simulink model "heatdrive_ecc_coupled_se21"  (R2025b)
settings: Solver=ode23t  StartTime=0.0  StopTime=10  FixedStep=0.1  MaxStep=0.4  RelTol=1e-2  AbsTol=1e-3
values from neighbouring files (symbols this model uses):
  cold_load_heat_W = 0.0    (= 0)    [Build_Simulink_Exchange_Params.m]
  cold_load_T_init = get_stage_field(stage_config, 'cold_load_T_in', get_stage_field(stage_config,          'chip_T_in', get_option_field(exchange_options, 'cold_load_T_init', get_option_field(exchange_options, 'chip_T_init', 293.0))))    [Build_Simulink_Exchange_Params.m]    (also in Create_Simulink_Exchange_Runtime.m = get_option_field(options, 'cold_load_T_init',          get_o)
  cold_sink_T_init = get_stage_field(stage_config, 'cold_sink_T_in', get_option_field(exchange_options, 'cold_sink_T_init', 293.0))    [Build_Simulink_Exchange_Params.m]    (also in Create_Simulink_Exchange_Runtime.m = get_option_field(options, 'cold_sink_T_init', ambient_T_init)
  hot_sink_T_init = get_stage_field(stage_config, 'hot_sink_T_in', get_option_field(exchange_options, 'hot_sink_T_init', 293.0))    [Build_Simulink_Exchange_Params.m]    (also in Create_Simulink_Exchange_Runtime.m = get_option_field(options, 'hot_sink_T_init', ambient_T_init))
  mdot_cooldown_source_kgps = mdot_target_kgps    [Build_Simulink_Exchange_Params.m]
  mdot_hold_source_kgps = mdot_target_kgps    [Build_Simulink_Exchange_Params.m]
  pressure_pi_bias_MPa = pressure_pi_dp_guess_MPa    [Build_Simulink_Exchange_Params.m]
  pressure_pi_error_filter_tau_s = max(get_option_field(exchange_options, 'pressure_pi_error_filter_tau_s', 0.002), 1.0e-5)    [Build_Simulink_Exchange_Params.m]
  pressure_pi_error_normalization_gain_kgps_inv = 1.0    (= 1)    [Build_Simulink_Exchange_Params.m]
  pressure_pi_max_MPa = pressure_pi_dp_guess_MPa + pressure_pi_margin_MPa    [Build_Simulink_Exchange_Params.m]
  shex_sink_T_init = get_option_field(exchange_options, 'shex_sink_T_init', hot_sink_T_init)    [Build_Simulink_Exchange_Params.m]
undefined symbols (not defined in the file or in its folder): constitutive_sample_time_s, constitutive_state21_initial, se_constitutive_T21_initial, se_pressure_integrator_max_MPa, se_pressure_pi_ki_MPa_per_kgps_s, se_pressure_pi_kp_MPa_per_kgps, se_pressure_pi_min_MPa, se_solver_T_init_21_internal, se_stage2_pressure_integrator_min_MPa, se_stage4_pressure_integrator_min_MPa, sma_constitutive_T21_initial, sma_mdot_stage1_source_kgps, sma_mdot_stage3_source_kgps, sma_pressure_integrator_max_MPa, sma_pressure_integrator_min_MPa, sma_pressure_pi_ki_MPa_per_kgps_s, sma_pressure_pi_kp_MPa_per_kgps, sma_pressure_pi_min_MPa, sma_solver_T_init_21_internal
libraries: fl_lib x484, nesl_utility x232, SimscapeFluids_lib x20
(part 1 of 8)
settings Model: Creator=Yanchenxi  LastModifiedBy=86182
settings RTWCC: GPUComputeCapability=3.5
settings SimscapeCC: ExplicitSolverDiagnosticOptions=none  SimscapeLogType=all  SimscapeLogSimulationStatistics=on  SimscapeLogToSDI=on

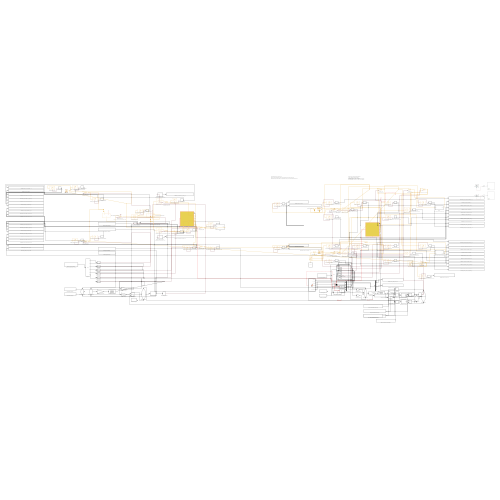
[thumbnail: Simulink's stored preview of the top-level diagram]
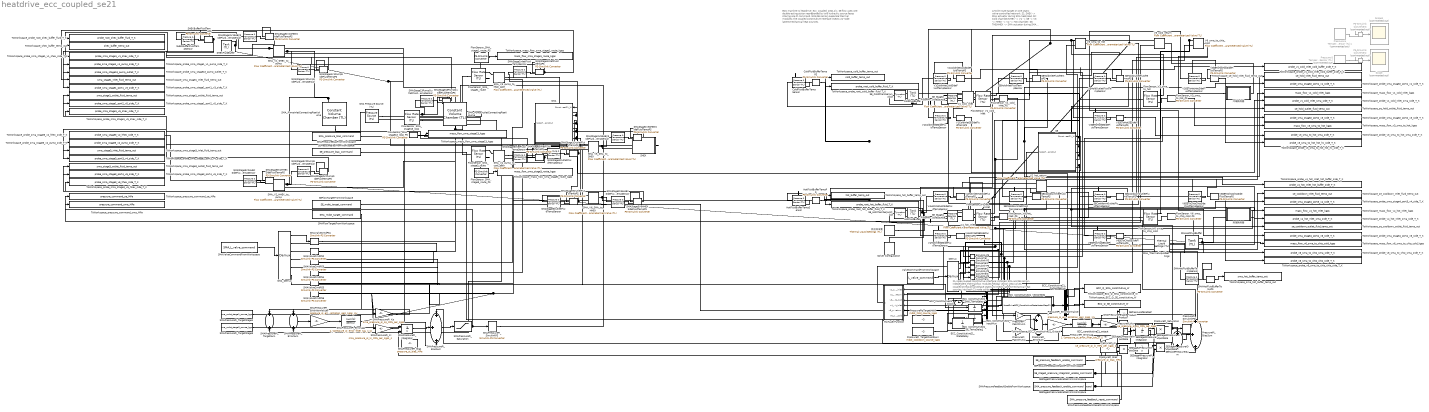
== system heatdrive_ecc_coupled_se21 ==
  note: ECC mainline is heatdrive_ecc_coupled_se21.slx.
      | SE flow uses one double-acting piston represented by two hydraulic source faces sharing one PI command.
      | SMA/SE remain separate thermal modules; the coupled constitutive interface injects 21-node latent/mechanical heat sources.
  note: Article route target on one static valve-controlled network:
      | S1: SHEX -> SMA actuator during SMA heat/load.
      | S2: Cold chamber/CHEX -> V1 -> SE -> V3 -> HHEX -> V2 -> Hot chamber.
      | S3: THE/HHEX -> SMA actuator during SMA cool/unload.
      | S4: Hot chamber/HHEX -> V4 -> SE -> V6 -> CHEX -> V5 -> Cold chamber.
  note: 21-node coupled constitutive interface installed.
      | SMA and SE remain independent thermal/flow modules.
      | Global vector step solves coupled stress/strain/phase state and injects latent/mechanical heat sources into both 21-node solids.
  ColdFluidBuffer : SimscapeFluids_lib/Thermal Liquid/Tanks & Accumulators/Tank (TL)  num_inlet=fluids.thermal_liquid.tanks_accumulators.enum.NumInlet.One  pressure_spec=fluids.thermal_liquid.tanks_accumulators.enum.TankPressureSpec.Specified  tank_pressure=tank_pressure_MPa MPa  volume_spec=fluids.thermal_liquid.tanks_accumulators.enum.TankVolumeSpec.Constant  tank_area=fluid_buffer_tank_area_m2 m^2  level_TLU=[0, 3, 5] m  volume_TLU=[0, 4, 6] m^3  inlet_height_A=0 m  inlet_area_A=0.01 m^2  inlet_heights_AB=[.1, .1] m  inlet_areas_AB=[.01, .01] m^2  inlet_heights_ABC=[.1, .1, .1] m  inlet_areas_ABC=[.01, .01, .01] m^2  inlet_heights_ABCD=0.1 * ones(1, 4) m  inlet_areas_ABCD=0.01 * ones(1, 4) m^2  inlet_heights_ABCDE=0.1 * ones(1, 5) m  inlet_areas_ABCDE=0.01 * ones(1, 5) m^2  inlet_heights_ABCDEF=0.1 * ones(1, 6) m  inlet_areas_ABCDEF=0.01 * ones(1, 6) m^2  level_check=simscape.enum.assert.action.error  capacity_check=simscape.enum.assert.action.none  max_capacity=fluid_buffer_max_capacity_m3 m^3  g=9.81 m/s^2  level_specify=on  level_priority=High  level=fluid_buffer_tank_level_m m  level_nominal_specify=off  level_nominal_value=1  level_nominal_unit=m  volume_specify=off  volume_priority=None  volume=5 m^3  volume_nominal_specify=off  volume_nominal_value=1  volume_nominal_unit=m^3  mass_specify=off  mass_priority=None  mass=5000 kg  mass_nominal_specify=off  mass_nominal_value=1  mass_nominal_unit=kg  T_I_specify=on  T_I_priority=High  T_I=cold_fluid_buffer_T_init K  T_I_nominal_specify=off  T_I_nominal_value=1  T_I_nominal_unit=K
      settings: InternalSimscapePortConfiguration="{\"Bottom\":[{\"id\":\"H\",\"label\":\"H\",\"type\":\"foundation.thermal.thermal\"},{\"id\":\"T_out\",\"label\":\"T\",\"type\":\"output\"}],\"Left\":[{\"id\":\"A\",\"label\":\"A\",\"type\":\"foundation.thermal_liquid.thermal_liquid\"}],\"Right\":[],\"Top\":[{\"id\":\"V_out\",\"label\":\"V\",\"type\":\"output\"},{\"id\":\"L_out\",\"label\":\"L\",\"type\":\"output\"}]}"
  ColdFluidBufferTempPS : nesl_utility/PS-Simulink Converter  PhysicalDomain=network_engine_domain  SubClassName=ps_output  LeftPortType=input  RightPortType=output  PseudoPeriodic=off  Frequencies=[]  VectorFormat=1-D array  Unit=K  AffineConversion=off
      settings: AttributesFormatString=CHEX exchanger retained from mature model
  ColdFluidBufferTempSensor : fl_lib/Thermal Liquid/Sensors/Pressure & Temperature Sensor (TL)  reference=foundation.enum.MeasurementReference.absolute  pressure=false  pressure_spec=foundation.enum.PressureMeasementSpec.Absolute  temperature=true
      settings: InternalSimscapePortConfiguration="{\"Bottom\":[{\"id\":\"T\",\"label\":\"T\",\"type\":\"output\"}],\"Left\":[{\"id\":\"A\",\"label\":\"A\",\"type\":\"foundation.thermal_liquid.thermal_liquid\"}],\"Right\":[],\"Top\":[]}"
  Demux : Demux  Outputs=6
      settings: DisplayOption=none
  ECC_Constitutive21_Clock : Clock
  ECC_Constitutive21_InputMux : Mux
  ECC_Constitutive21_OutputDemux : Demux  Outputs=[21 21 210]
  ECC_Constitutive21_SE_TempDelay : UnitDelay  InitialCondition=se_constitutive_T21_initial  SampleTime=constitutive_sample_time_s  HasFrameUpgradeWarning=on
  ECC_Constitutive21_SMA_TempDelay : UnitDelay  InitialCondition=sma_constitutive_T21_initial  SampleTime=constitutive_sample_time_s  HasFrameUpgradeWarning=on
  ECC_Constitutive21_StateDelay : UnitDelay  InitialCondition=constitutive_state21_initial  SampleTime=constitutive_sample_time_s  HasFrameUpgradeWarning=on
  ECC_Constitutive21_VectorStep : MATLABFcn  MATLABFcn=HeatDriveECC_ConstitutiveStateVectorStep21  OutputDimensions=252  SampleTime=constitutive_sample_time_s
  FlowSensor_SMA_stage13_loop : fl_lib/Thermal Liquid/Sensors/Flow Rate Sensor (TL)  mass_flow_measure=true  volumetric_flow_measure=false  energy_flow_measure=false
      settings: InternalSimscapePortConfiguration="{\"Bottom\":[],\"Left\":[{\"id\":\"A\",\"label\":\"A\",\"type\":\"foundation.thermal_liquid.thermal_liquid\"}],\"Right\":[{\"id\":\"B\",\"label\":\"B\",\"type\":\"foundation.thermal_liquid.thermal_liquid\"},{\"id\":\"M\",\"label\":\"M\",\"type\":\"output\"}],\"Top\":[]}"
  FlowSensor_SMA_stage13_loop_PS : nesl_utility/PS-Simulink Converter  PhysicalDomain=network_engine_domain  SubClassName=ps_output  LeftPortType=input  RightPortType=output  PseudoPeriodic=off  Frequencies=[]  VectorFormat=1-D array  Unit=kg/s  AffineConversion=off
      settings: AttributesFormatString=CHEX exchanger retained from mature model
  FlowSensor_SMA_stage1_route : fl_lib/Thermal Liquid/Sensors/Flow Rate Sensor (TL)  mass_flow_measure=true  volumetric_flow_measure=false  energy_flow_measure=false
      settings: InternalSimscapePortConfiguration="{\"Bottom\":[],\"Left\":[{\"id\":\"A\",\"label\":\"A\",\"type\":\"foundation.thermal_liquid.thermal_liquid\"}],\"Right\":[{\"id\":\"B\",\"label\":\"B\",\"type\":\"foundation.thermal_liquid.thermal_liquid\"},{\"id\":\"M\",\"label\":\"M\",\"type\":\"output\"}],\"Top\":[]}"
  FlowSensor_SMA_stage1_route_PS : nesl_utility/PS-Simulink Converter  PhysicalDomain=network_engine_domain  SubClassName=ps_output  LeftPortType=input  RightPortType=output  PseudoPeriodic=off  Frequencies=[]  VectorFormat=1-D array  Unit=kg/s  AffineConversion=off
      settings: AttributesFormatString=CHEX exchanger retained from mature model
  FlowSensor_SMA_stage3_route : fl_lib/Thermal Liquid/Sensors/Flow Rate Sensor (TL)  mass_flow_measure=true  volumetric_flow_measure=false  energy_flow_measure=false
      settings: InternalSimscapePortConfiguration="{\"Bottom\":[],\"Left\":[{\"id\":\"A\",\"label\":\"A\",\"type\":\"foundation.thermal_liquid.thermal_liquid\"}],\"Right\":[{\"id\":\"B\",\"label\":\"B\",\"type\":\"foundation.thermal_liquid.thermal_liquid\"},{\"id\":\"M\",\"label\":\"M\",\"type\":\"output\"}],\"Top\":[]}"
  FlowSensor_SMA_stage3_route_PS : nesl_utility/PS-Simulink Converter  PhysicalDomain=network_engine_domain  SubClassName=ps_output  LeftPortType=input  RightPortType=output  PseudoPeriodic=off  Frequencies=[]  VectorFormat=1-D array  Unit=kg/s  AffineConversion=off
      settings: AttributesFormatString=CHEX exchanger retained from mature model
  FlowSensor_V1_cold_inlet : fl_lib/Thermal Liquid/Sensors/Flow Rate Sensor (TL)  mass_flow_measure=true  volumetric_flow_measure=false  energy_flow_measure=false
      settings: InternalSimscapePortConfiguration="{\"Bottom\":[],\"Left\":[{\"id\":\"A\",\"label\":\"A\",\"type\":\"foundation.thermal_liquid.thermal_liquid\"}],\"Right\":[{\"id\":\"B\",\"label\":\"B\",\"type\":\"foundation.thermal_liquid.thermal_liquid\"},{\"id\":\"M\",\"label\":\"M\",\"type\":\"output\"}],\"Top\":[]}"
  FlowSensor_V1_cold_inlet_PS : nesl_utility/PS-Simulink Converter  PhysicalDomain=network_engine_domain  SubClassName=ps_output  LeftPortType=input  RightPortType=output  PseudoPeriodic=off  Frequencies=[]  VectorFormat=1-D array  Unit=kg/s  AffineConversion=off
      settings: AttributesFormatString=CHEX exchanger retained from mature model
  FlowSensor_V3_sma_to_hot : fl_lib/Thermal Liquid/Sensors/Flow Rate Sensor (TL)  mass_flow_measure=true  volumetric_flow_measure=false  energy_flow_measure=false
      settings: InternalSimscapePortConfiguration="{\"Bottom\":[],\"Left\":[{\"id\":\"A\",\"label\":\"A\",\"type\":\"foundation.thermal_liquid.thermal_liquid\"}],\"Right\":[{\"id\":\"B\",\"label\":\"B\",\"type\":\"foundation.thermal_liquid.thermal_liquid\"},{\"id\":\"M\",\"label\":\"M\",\"type\":\"output\"}],\"Top\":[]}"
  FlowSensor_V3_sma_to_hot_PS : nesl_utility/PS-Simulink Converter  PhysicalDomain=network_engine_domain  SubClassName=ps_output  LeftPortType=input  RightPortType=output  PseudoPeriodic=off  Frequencies=[]  VectorFormat=1-D array  Unit=kg/s  AffineConversion=off
      settings: AttributesFormatString=HHEX/THE exchanger retained from mature model
  FlowSensor_V4_hot_inlet : fl_lib/Thermal Liquid/Sensors/Flow Rate Sensor (TL)  mass_flow_measure=true  volumetric_flow_measure=false  energy_flow_measure=false
      settings: InternalSimscapePortConfiguration="{\"Bottom\":[],\"Left\":[{\"id\":\"A\",\"label\":\"A\",\"type\":\"foundation.thermal_liquid.thermal_liquid\"}],\"Right\":[{\"id\":\"B\",\"label\":\"B\",\"type\":\"foundation.thermal_liquid.thermal_liquid\"},{\"id\":\"M\",\"label\":\"M\",\"type\":\"output\"}],\"Top\":[]}"
  FlowSensor_V4_hot_inlet_PS : nesl_utility/PS-Simulink Converter  PhysicalDomain=network_engine_domain  SubClassName=ps_output  LeftPortType=input  RightPortType=output  PseudoPeriodic=off  Frequencies=[]  VectorFormat=1-D array  Unit=kg/s  AffineConversion=off
      settings: AttributesFormatString=HHEX/THE exchanger retained from mature model
  FlowSensor_V6_sma_to_chip_cold : fl_lib/Thermal Liquid/Sensors/Flow Rate Sensor (TL)  mass_flow_measure=true  volumetric_flow_measure=false  energy_flow_measure=false
      settings: InternalSimscapePortConfiguration="{\"Bottom\":[],\"Left\":[{\"id\":\"A\",\"label\":\"A\",\"type\":\"foundation.thermal_liquid.thermal_liquid\"}],\"Right\":[{\"id\":\"B\",\"label\":\"B\",\"type\":\"foundation.thermal_liquid.thermal_liquid\"},{\"id\":\"M\",\"label\":\"M\",\"type\":\"output\"}],\"Top\":[]}"
  FlowSensor_V6_sma_to_chip_cold_PS : nesl_utility/PS-Simulink Converter  PhysicalDomain=network_engine_domain  SubClassName=ps_output  LeftPortType=input  RightPortType=output  PseudoPeriodic=off  Frequencies=[]  VectorFormat=1-D array  Unit=kg/s  AffineConversion=off
      settings: AttributesFormatString=CHEX exchanger retained from mature model
  HotFluidBuffer : SimscapeFluids_lib/Thermal Liquid/Tanks & Accumulators/Tank (TL)  num_inlet=fluids.thermal_liquid.tanks_accumulators.enum.NumInlet.One  pressure_spec=fluids.thermal_liquid.tanks_accumulators.enum.TankPressureSpec.Specified  tank_pressure=tank_pressure_MPa MPa  volume_spec=fluids.thermal_liquid.tanks_accumulators.enum.TankVolumeSpec.Constant  tank_area=fluid_buffer_tank_area_m2 m^2  level_TLU=[0, 3, 5] m  volume_TLU=[0, 4, 6] m^3  inlet_height_A=0 m  inlet_area_A=0.01 m^2  inlet_heights_AB=[.1, .1] m  inlet_areas_AB=[.01, .01] m^2  inlet_heights_ABC=[.1, .1, .1] m  inlet_areas_ABC=[.01, .01, .01] m^2  inlet_heights_ABCD=0.1 * ones(1, 4) m  inlet_areas_ABCD=0.01 * ones(1, 4) m^2  inlet_heights_ABCDE=0.1 * ones(1, 5) m  inlet_areas_ABCDE=0.01 * ones(1, 5) m^2  inlet_heights_ABCDEF=0.1 * ones(1, 6) m  inlet_areas_ABCDEF=0.01 * ones(1, 6) m^2  level_check=simscape.enum.assert.action.error  capacity_check=simscape.enum.assert.action.none  max_capacity=fluid_buffer_max_capacity_m3 m^3  g=9.81 m/s^2  level_specify=on  level_priority=High  level=fluid_buffer_tank_level_m m  level_nominal_specify=off  level_nominal_value=1  level_nominal_unit=m  volume_specify=off  volume_priority=None  volume=5 m^3  volume_nominal_specify=off  volume_nominal_value=1  volume_nominal_unit=m^3  mass_specify=off  mass_priority=None  mass=5000 kg  mass_nominal_specify=off  mass_nominal_value=1  mass_nominal_unit=kg  T_I_specify=on  T_I_priority=High  T_I=hot_fluid_buffer_T_init K  T_I_nominal_specify=off  T_I_nominal_value=1  T_I_nominal_unit=K
      settings: InternalSimscapePortConfiguration="{\"Bottom\":[{\"id\":\"H\",\"label\":\"H\",\"type\":\"foundation.thermal.thermal\"},{\"id\":\"T_out\",\"label\":\"T\",\"type\":\"output\"}],\"Left\":[{\"id\":\"A\",\"label\":\"A\",\"type\":\"foundation.thermal_liquid.thermal_liquid\"}],\"Right\":[],\"Top\":[{\"id\":\"V_out\",\"label\":\"V\",\"type\":\"output\"},{\"id\":\"L_out\",\"label\":\"L\",\"type\":\"output\"}]}"
  HotFluidBufferTempPS : nesl_utility/PS-Simulink Converter  PhysicalDomain=network_engine_domain  SubClassName=ps_output  LeftPortType=input  RightPortType=output  PseudoPeriodic=off  Frequencies=[]  VectorFormat=1-D array  Unit=K  AffineConversion=off
      settings: AttributesFormatString=HHEX/THE exchanger retained from mature model
  HotFluidBufferTempSensor : fl_lib/Thermal Liquid/Sensors/Pressure & Temperature Sensor (TL)  reference=foundation.enum.MeasurementReference.absolute  pressure=false  pressure_spec=foundation.enum.PressureMeasementSpec.Absolute  temperature=true
      settings: InternalSimscapePortConfiguration="{\"Bottom\":[{\"id\":\"T\",\"label\":\"T\",\"type\":\"output\"}],\"Left\":[{\"id\":\"A\",\"label\":\"A\",\"type\":\"foundation.thermal_liquid.thermal_liquid\"}],\"Right\":[],\"Top\":[]}"
  MATLAB Function : MATLAB Function  TreatAsAtomicUnit=on
  PS-Simulink Converter2 : nesl_utility/PS-Simulink Converter  Commented=on  PhysicalDomain=network_engine_domain  SubClassName=ps_output  LeftPortType=input  RightPortType=output  PseudoPeriodic=off  Frequencies=[]  VectorFormat=1-D array  Unit=1  AffineConversion=off
  PS-Simulink Converter3 : nesl_utility/PS-Simulink Converter  Commented=on  PhysicalDomain=network_engine_domain  SubClassName=ps_output  LeftPortType=input  RightPortType=output  PseudoPeriodic=off  Frequencies=[]  VectorFormat=1-D array  Unit=1  AffineConversion=off
  Pressure & Temperature Sensor (TL) : fl_lib/Thermal Liquid/Sensors/Pressure & Temperature Sensor (TL)  Commented=on  reference=foundation.enum.MeasurementReference.absolute  pressure=false  pressure_spec=foundation.enum.PressureMeasementSpec.Absolute  temperature=true
      settings: InternalSimscapePortConfiguration="{\"Bottom\":[{\"id\":\"T\",\"label\":\"T\",\"type\":\"output\"}],\"Left\":[{\"id\":\"A\",\"label\":\"A\",\"type\":\"foundation.thermal_liquid.thermal_liquid\"}],\"Right\":[],\"Top\":[]}"
  Pressure & Temperature Sensor (TL)1 : fl_lib/Thermal Liquid/Sensors/Pressure & Temperature Sensor (TL)  Commented=on  reference=foundation.enum.MeasurementReference.absolute  pressure=false  pressure_spec=foundation.enum.PressureMeasementSpec.Absolute  temperature=true
      settings: InternalSimscapePortConfiguration="{\"Bottom\":[{\"id\":\"T\",\"label\":\"T\",\"type\":\"output\"}],\"Left\":[{\"id\":\"A\",\"label\":\"A\",\"type\":\"foundation.thermal_liquid.thermal_liquid\"}],\"Right\":[],\"Top\":[]}"
  PressurePI_Bias : Constant  Value=pressure_pi_bias_MPa
  PressurePI_BiasSum : Sum  Inputs=+++
  PressurePI_ErrorLag : TransferFcn  Numerator=1  Denominator=[pressure_pi_error_filter_tau_s 1]
  PressurePI_ErrorNormalizer : Gain  Gain=pressure_pi_error_normalization_gain_kgps_inv
  PressurePI_ErrorSum : Sum  Inputs=++--
  PressurePI_Ki : Gain  Gain=se_pressure_pi_ki_MPa_per_kgps_s
  PressurePI_Kp : Gain  Gain=se_pressure_pi_kp_MPa_per_kgps
  PressurePI_PassthruV1 : Gain
  PressurePI_PassthruV4 : Gain
  PressurePI_Saturation : Saturate  UpperLimit=pressure_pi_max_MPa  LowerLimit=se_pressure_pi_min_MPa
  PressurePI_SimulinkPS : nesl_utility/Simulink-PS Converter  PhysicalDomain=network_engine_domain  SubClassName=ps_input  LeftPortType=input  RightPortType=output  PseudoPeriodic=off  Frequencies=[]  NoiseDistribution=none  NoiseParameters=[]  Unit=MPa  AffineConversion=off  FilteringAndDerivatives=provide  SimscapeFilterOrder=1  InputFilterTimeConstant=0.001  UdotUserProvided=0
  PressurePI_TargetCooldown : Constant  Value=mdot_cooldown_source_kgps
  PressurePI_TargetHold : Constant  Value=mdot_hold_source_kgps
  SE : Subsystem
      settings: AttributesFormatString=Active dual-path SE21 exchanger shell; ECC solid law is handled separately
  SECooldownInletFluidTempPS : nesl_utility/PS-Simulink Converter  PhysicalDomain=network_engine_domain  SubClassName=ps_output  LeftPortType=input  RightPortType=output  PseudoPeriodic=off  Frequencies=[]  VectorFormat=1-D array  Unit=K  AffineConversion=off
  SECooldownInletFluidTempSensor : fl_lib/Thermal Liquid/Sensors/Pressure & Temperature Sensor (TL)  reference=foundation.enum.MeasurementReference.absolute  pressure=false  pressure_spec=foundation.enum.PressureMeasementSpec.Absolute  temperature=true
      settings: InternalSimscapePortConfiguration="{\"Bottom\":[{\"id\":\"T\",\"label\":\"T\",\"type\":\"output\"}],\"Left\":[{\"id\":\"A\",\"label\":\"A\",\"type\":\"foundation.thermal_liquid.thermal_liquid\"}],\"Right\":[],\"Top\":[]}"
  SECooldownOutletFluidTempPS : nesl_utility/PS-Simulink Converter  PhysicalDomain=network_engine_domain  SubClassName=ps_output  LeftPortType=input  RightPortType=output  PseudoPeriodic=off  Frequencies=[]  VectorFormat=1-D array  Unit=K  AffineConversion=off
  SECooldownOutletFluidTempSensor : fl_lib/Thermal Liquid/Sensors/Pressure & Temperature Sensor (TL)  reference=foundation.enum.MeasurementReference.absolute  pressure=false  pressure_spec=foundation.enum.PressureMeasementSpec.Absolute  temperature=true
      settings: InternalSimscapePortConfiguration="{\"Bottom\":[{\"id\":\"T\",\"label\":\"T\",\"type\":\"output\"}],\"Left\":[{\"id\":\"A\",\"label\":\"A\",\"type\":\"foundation.thermal_liquid.thermal_liquid\"}],\"Right\":[],\"Top\":[]}"
  SEFlowTargetFromWorkspace : FromWorkspace  VariableName=SE_mdot_target_command  OutputAfterFinalValue=Holding final value
  SEHoldInletFluidTempPS : nesl_utility/PS-Simulink Converter  PhysicalDomain=network_engine_domain  SubClassName=ps_output  LeftPortType=input  RightPortType=output  PseudoPeriodic=off  Frequencies=[]  VectorFormat=1-D array  Unit=K  AffineConversion=off
  SEHoldInletFluidTempSensor : fl_lib/Thermal Liquid/Sensors/Pressure & Temperature Sensor (TL)  reference=foundation.enum.MeasurementReference.absolute  pressure=false  pressure_spec=foundation.enum.PressureMeasementSpec.Absolute  temperature=true
      settings: InternalSimscapePortConfiguration="{\"Bottom\":[{\"id\":\"T\",\"label\":\"T\",\"type\":\"output\"}],\"Left\":[{\"id\":\"A\",\"label\":\"A\",\"type\":\"foundation.thermal_liquid.thermal_liquid\"}],\"Right\":[],\"Top\":[]}"
  SEHoldOutletFluidTempPS : nesl_utility/PS-Simulink Converter  PhysicalDomain=network_engine_domain  SubClassName=ps_output  LeftPortType=input  RightPortType=output  PseudoPeriodic=off  Frequencies=[]  VectorFormat=1-D array  Unit=K  AffineConversion=off
  SEHoldOutletFluidTempSensor : fl_lib/Thermal Liquid/Sensors/Pressure & Temperature Sensor (TL)  reference=foundation.enum.MeasurementReference.absolute  pressure=false  pressure_spec=foundation.enum.PressureMeasementSpec.Absolute  temperature=true
      settings: InternalSimscapePortConfiguration="{\"Bottom\":[{\"id\":\"T\",\"label\":\"T\",\"type\":\"output\"}],\"Left\":[{\"id\":\"A\",\"label\":\"A\",\"type\":\"foundation.thermal_liquid.thermal_liquid\"}],\"Right\":[],\"Top\":[]}"
  SEPressureBiasFromWorkspace : FromWorkspace  VariableName=SE_pressure_bias_command  OutputAfterFinalValue=Holding final value
  SEPressureFeedbackEnableFromWorkspace : FromWorkspace  VariableName=SE_pressure_feedback_enable_command  Interpolate=off  OutputAfterFinalValue=Holding final value
  SEPressurePEnableProduct : Product  Inputs=**
  SERoutePressureISum : Sum
  SEStage2PressureIEnableFromWorkspace : FromWorkspace  VariableName=SE_stage2_pressure_integrator_enable_command  Interpolate=off  OutputAfterFinalValue=Holding final value
  SEStage2PressureIInputGate : Product  Inputs=**
  SEStage2PressureIOutputGate : Product  Inputs=**
  SEStage2PressurePI_Integrator : Integrator  LimitOutput=on  UpperSaturationLimit=se_pressure_integrator_max_MPa  LowerSaturationLimit=se_stage2_pressure_integrator_min_MPa
  SEStage4PressureIEnableFromWorkspace : FromWorkspace  VariableName=SE_stage4_pressure_integrator_enable_command  Interpolate=off  OutputAfterFinalValue=Holding final value
  SEStage4PressureIInputGate : Product  Inputs=**
  SEStage4PressureIOutputGate : Product  Inputs=**
  SEStage4PressurePI_Integrator : Integrator  LimitOutput=on  UpperSaturationLimit=se_pressure_integrator_max_MPa  LowerSaturationLimit=se_stage4_pressure_integrator_min_MPa
  SE_ColdChamberJunction : SimscapeFluids_lib/Thermal Liquid/Pipes & Fittings/T-Junction (TL)  area_main=pipe_fa m^2  area_branch=pipe_fa m^2  junction_spec=fluids.thermal_liquid.pipes_fittings.enum.TLossCoefficientModel.Crane  k_main_converge=1.12  k_main_diverge=1.12  k_branch_converge=1.12  k_branch_diverge=1.12  loss_coeff_A=1  loss_coeff_B=1  loss_coeff_C=1  radius=0.001 m  Re_c=150  Re_0=10  tau=0.0001 s  saturation_ratio=0.2  smoothing_factor=0.01  inertia=false
      settings: InternalSimscapePortConfiguration="{\"Bottom\":[{\"id\":\"C\",\"label\":\"C\",\"type\":\"foundation.thermal_liquid.thermal_liquid\"}],\"Left\":[{\"id\":\"A\",\"label\":\"A\",\"type\":\"foundation.thermal_liquid.thermal_liquid\"}],\"Right\":[{\"id\":\"B\",\"label\":\"B\",\"type\":\"foundation.thermal_liquid.thermal_liquid\"}],\"Top\":[]}"
  SE_HotChamberJunction : SimscapeFluids_lib/Thermal Liquid/Pipes & Fittings/T-Junction (TL)  area_main=0.01 m^2  area_branch=0.01 m^2  junction_spec=fluids.thermal_liquid.pipes_fittings.enum.TLossCoefficientModel.Crane  k_main_converge=1.12  k_main_diverge=1.12  k_branch_converge=1.12  k_branch_diverge=1.12  loss_coeff_A=1  loss_coeff_B=1  loss_coeff_C=1  radius=0.001 m  Re_c=150  Re_0=10  tau=0.0001 s  saturation_ratio=0.2  smoothing_factor=0.01  inertia=false
      settings: InternalSimscapePortConfiguration="{\"Bottom\":[{\"id\":\"C\",\"label\":\"C\",\"type\":\"foundation.thermal_liquid.thermal_liquid\"}],\"Left\":[{\"id\":\"A\",\"label\":\"A\",\"type\":\"foundation.thermal_liquid.thermal_liquid\"}],\"Right\":[{\"id\":\"B\",\"label\":\"B\",\"type\":\"foundation.thermal_liquid.thermal_liquid\"}],\"Top\":[]}"
  SE_Stage2_PistonPressureSource : fl_lib/Thermal Liquid/Sources/Pressure Source (TL)  source_type=foundation.enum.constant_controlled.controlled  pressure_differential=pressure_differential_MPa MPa  power_spec=foundation.enum.power_spec.none  area=pipe_fa m^2
      settings: AttributesFormatString=Stage 2 hydraulic face of the single SE double-acting piston  InternalSimscapePortConfiguration="{\"Bottom\":[],\"Left\":[{\"id\":\"A\",\"label\":\"A\",\"type\":\"foundation.thermal_liquid.thermal_liquid\"},{\"id\":\"P\",\"label\":\"P\",\"type\":\"input\"}],\"Right\":[{\"id\":\"B\",\"label\":\"B\",\"type\":\"foundation.thermal_liquid.thermal_liquid\"}],\"Top\":[]}"
  SE_Stage4_PistonPressureSource : fl_lib/Thermal Liquid/Sources/Pressure Source (TL)  source_type=foundation.enum.constant_controlled.controlled  pressure_differential=pressure_differential_MPa MPa  power_spec=foundation.enum.power_spec.none  area=pipe_fa m^2
      settings: AttributesFormatString=Stage 4 hydraulic face of the single SE double-acting piston  InternalSimscapePortConfiguration="{\"Bottom\":[],\"Left\":[{\"id\":\"A\",\"label\":\"A\",\"type\":\"foundation.thermal_liquid.thermal_liquid\"},{\"id\":\"P\",\"label\":\"P\",\"type\":\"input\"}],\"Right\":[{\"id\":\"B\",\"label\":\"B\",\"type\":\"foundation.thermal_liquid.thermal_liquid\"}],\"Top\":[]}"
  SHEX : Subsystem
  SHEXBufferFluidTempPS : nesl_utility/PS-Simulink Converter  PhysicalDomain=network_engine_domain  SubClassName=ps_output  LeftPortType=input  RightPortType=output  PseudoPeriodic=off  Frequencies=[]  VectorFormat=1-D array  Unit=K  AffineConversion=off
  SHEXBufferFluidTempSensor : fl_lib/Thermal Liquid/Sensors/Pressure & Temperature Sensor (TL)  reference=foundation.enum.MeasurementReference.absolute  pressure=false  pressure_spec=foundation.enum.PressureMeasementSpec.Absolute  temperature=true
      settings: InternalSimscapePortConfiguration="{\"Bottom\":[{\"id\":\"T\",\"label\":\"T\",\"type\":\"output\"}],\"Left\":[{\"id\":\"A\",\"label\":\"A\",\"type\":\"foundation.thermal_liquid.thermal_liquid\"}],\"Right\":[],\"Top\":[]}"
  SHEXFluidBuffer : SimscapeFluids_lib/Thermal Liquid/Tanks & Accumulators/Tank (TL)  num_inlet=fluids.thermal_liquid.tanks_accumulators.enum.NumInlet.One  pressure_spec=fluids.thermal_liquid.tanks_accumulators.enum.TankPressureSpec.Specified  tank_pressure=tank_pressure_MPa MPa  volume_spec=fluids.thermal_liquid.tanks_accumulators.enum.TankVolumeSpec.Constant  tank_area=fluid_buffer_tank_area_m2 m^2  level_TLU=[0, 3, 5] m  volume_TLU=[0, 4, 6] m^3  inlet_height_A=0 m  inlet_area_A=0.01 m^2  inlet_heights_AB=[.1, .1] m  inlet_areas_AB=[.01, .01] m^2  inlet_heights_ABC=[.1, .1, .1] m  inlet_areas_ABC=[.01, .01, .01] m^2  inlet_heights_ABCD=0.1 * ones(1, 4) m  inlet_areas_ABCD=0.01 * ones(1, 4) m^2  inlet_heights_ABCDE=0.1 * ones(1, 5) m  inlet_areas_ABCDE=0.01 * ones(1, 5) m^2  inlet_heights_ABCDEF=0.1 * ones(1, 6) m  inlet_areas_ABCDEF=0.01 * ones(1, 6) m^2  level_check=simscape.enum.assert.action.error  capacity_check=simscape.enum.assert.action.none  max_capacity=fluid_buffer_max_capacity_m3 m^3  g=9.81 m/s^2  level_specify=on  level_priority=High  level=fluid_buffer_tank_level_m m  level_nominal_specify=off  level_nominal_value=1  level_nominal_unit=m  volume_specify=off  volume_priority=None  volume=5 m^3  volume_nominal_specify=off  volume_nominal_value=1  volume_nominal_unit=m^3  mass_specify=off  mass_priority=None  mass=5000 kg  mass_nominal_specify=off  mass_nominal_value=1  mass_nominal_unit=kg  T_I_specify=on  T_I_priority=High  T_I=shex_fluid_buffer_T_init K  T_I_nominal_specify=off  T_I_nominal_value=1  T_I_nominal_unit=K
      settings: InternalSimscapePortConfiguration="{\"Bottom\":[{\"id\":\"H\",\"label\":\"H\",\"type\":\"foundation.thermal.thermal\"},{\"id\":\"T_out\",\"label\":\"T\",\"type\":\"output\"}],\"Left\":[{\"id\":\"A\",\"label\":\"A\",\"type\":\"foundation.thermal_liquid.thermal_liquid\"}],\"Right\":[],\"Top\":[{\"id\":\"V_out\",\"label\":\"V\",\"type\":\"output\"},{\"id\":\"L_out\",\"label\":\"L\",\"type\":\"output\"}]}"
  SMA : Subsystem
  SMA Pressure Source (TL) : fl_lib/Thermal Liquid/Sources/Pressure Source (TL)  source_type=foundation.enum.constant_controlled.controlled  pressure_differential=pressure_differential_MPa MPa  power_spec=foundation.enum.power_spec.none  area=sma_pipe_fa m^2
      settings: AttributesFormatString=ECC pump / pressure source retained from mature model  InternalSimscapePortConfiguration="{\"Bottom\":[],\"Left\":[{\"id\":\"A\",\"label\":\"A\",\"type\":\"foundation.thermal_liquid.thermal_liquid\"},{\"id\":\"P\",\"label\":\"P\",\"type\":\"input\"}],\"Right\":[{\"id\":\"B\",\"label\":\"B\",\"type\":\"foundation.thermal_liquid.thermal_liquid\"}],\"Top\":[]}"
  SMAFlowTargetFromWorkspace : FromWorkspace  VariableName=SMA_mdot_target_command  OutputAfterFinalValue=Holding final value
  SMAHotFluidBuffer : SimscapeFluids_lib/Thermal Liquid/Tanks & Accumulators/Tank (TL)  num_inlet=fluids.thermal_liquid.tanks_accumulators.enum.NumInlet.One  pressure_spec=fluids.thermal_liquid.tanks_accumulators.enum.TankPressureSpec.Specified  tank_pressure=tank_pressure_MPa MPa  volume_spec=fluids.thermal_liquid.tanks_accumulators.enum.TankVolumeSpec.Constant  tank_area=fluid_buffer_tank_area_m2 m^2  level_TLU=[0, 3, 5] m  volume_TLU=[0, 4, 6] m^3  inlet_height_A=0 m  inlet_area_A=0.01 m^2  inlet_heights_AB=[.1, .1] m  inlet_areas_AB=[.01, .01] m^2  inlet_heights_ABC=[.1, .1, .1] m  inlet_areas_ABC=[.01, .01, .01] m^2  inlet_heights_ABCD=0.1 * ones(1, 4) m  inlet_areas_ABCD=0.01 * ones(1, 4) m^2  inlet_heights_ABCDE=0.1 * ones(1, 5) m  inlet_areas_ABCDE=0.01 * ones(1, 5) m^2  inlet_heights_ABCDEF=0.1 * ones(1, 6) m  inlet_areas_ABCDEF=0.01 * ones(1, 6) m^2  level_check=simscape.enum.assert.action.error  capacity_check=simscape.enum.assert.action.none  max_capacity=fluid_buffer_max_capacity_m3 m^3  g=9.81 m/s^2  level_specify=on  level_priority=High  level=fluid_buffer_tank_level_m m  level_nominal_specify=off  level_nominal_value=1  level_nominal_unit=m  volume_specify=off  volume_priority=None  volume=5 m^3  volume_nominal_specify=off  volume_nominal_value=1  volume_nominal_unit=m^3  mass_specify=off  mass_priority=None  mass=5000 kg  mass_nominal_specify=off  mass_nominal_value=1  mass_nominal_unit=kg  T_I_specify=on  T_I_priority=High  T_I=hot_fluid_buffer_T_init K  T_I_nominal_specify=off  T_I_nominal_value=1  T_I_nominal_unit=K
      settings: InternalSimscapePortConfiguration="{\"Bottom\":[{\"id\":\"H\",\"label\":\"H\",\"type\":\"foundation.thermal.thermal\"},{\"id\":\"T_out\",\"label\":\"T\",\"type\":\"output\"}],\"Left\":[{\"id\":\"A\",\"label\":\"A\",\"type\":\"foundation.thermal_liquid.thermal_liquid\"}],\"Right\":[],\"Top\":[{\"id\":\"V_out\",\"label\":\"V\",\"type\":\"output\"},{\"id\":\"L_out\",\"label\":\"L\",\"type\":\"output\"}]}"
  SMAHotFluidBufferTempPS : nesl_utility/PS-Simulink Converter  PhysicalDomain=network_engine_domain  SubClassName=ps_output  LeftPortType=input  RightPortType=output  PseudoPeriodic=off  Frequencies=[]  VectorFormat=1-D array  Unit=K  AffineConversion=off
      settings: AttributesFormatString=HHEX/THE exchanger retained from mature model
  SMAHotFluidBufferTempSensor : fl_lib/Thermal Liquid/Sensors/Pressure & Temperature Sensor (TL)  reference=foundation.enum.MeasurementReference.absolute  pressure=false  pressure_spec=foundation.enum.PressureMeasementSpec.Absolute  temperature=true
      settings: InternalSimscapePortConfiguration="{\"Bottom\":[{\"id\":\"T\",\"label\":\"T\",\"type\":\"output\"}],\"Left\":[{\"id\":\"A\",\"label\":\"A\",\"type\":\"foundation.thermal_liquid.thermal_liquid\"}],\"Right\":[],\"Top\":[]}"
  SMAPressureBiasFromWorkspace : FromWorkspace  VariableName=SMA_pressure_bias_command  OutputAfterFinalValue=Holding final value
  SMAPressureFeedbackEnableFromWorkspace : FromWorkspace  VariableName=SMA_pressure_feedback_enable_command  Interpolate=off  OutputAfterFinalValue=Holding final value
  SMAPressureFeedbackResetFromWorkspace : FromWorkspace  VariableName=SMA_pressure_feedback_reset_command  Interpolate=off  OutputAfterFinalValue=Holding final value
  SMAPressurePEnableProduct : Product  Inputs=**
  SMAPressurePI_Bias : Constant  Value=pressure_pi_bias_MPa
  SMAPressurePI_BiasSum : Sum  Inputs=+++
  SMAPressurePI_ErrorLag : TransferFcn  Numerator=1  Denominator=[pressure_pi_error_filter_tau_s 1]
  SMAPressurePI_ErrorNormalizer : Gain  Gain=pressure_pi_error_normalization_gain_kgps_inv
  SMAPressurePI_ErrorSum : Sum
  SMAPressurePI_Integrator : Integrator  ExternalReset=level  LimitOutput=on  UpperSaturationLimit=sma_pressure_integrator_max_MPa  LowerSaturationLimit=sma_pressure_integrator_min_MPa
  SMAPressurePI_Ki : Gain  Gain=sma_pressure_pi_ki_MPa_per_kgps_s
  SMAPressurePI_Kp : Gain  Gain=sma_pressure_pi_kp_MPa_per_kgps
  SMAPressurePI_Saturation : Saturate  UpperLimit=pressure_pi_max_MPa  LowerLimit=sma_pressure_pi_min_MPa
  SMAPressurePI_SimulinkPS : nesl_utility/Simulink-PS Converter  PhysicalDomain=network_engine_domain  SubClassName=ps_input  LeftPortType=input  RightPortType=output  PseudoPeriodic=off  Frequencies=[]  NoiseDistribution=none  NoiseParameters=[]  Unit=MPa  AffineConversion=off  FilteringAndDerivatives=provide  SimscapeFilterOrder=1  InputFilterTimeConstant=0.001  UdotUserProvided=0
  SMAPressurePI_TargetStage1 : Constant  Value=sma_mdot_stage1_source_kgps
  SMAPressurePI_TargetStage3 : Constant  Value=sma_mdot_stage3_source_kgps
  SMAPressurePI_TargetSum : Sum
  SMAStage13PumpOutletFluidTempPS : nesl_utility/PS-Simulink Converter  PhysicalDomain=network_engine_domain  SubClassName=ps_output  LeftPortType=input  RightPortType=output  PseudoPeriodic=off  Frequencies=[]  VectorFormat=1-D array  Unit=K  AffineConversion=off
  SMAStage13PumpOutletFluidTempSensor : fl_lib/Thermal Liquid/Sensors/Pressure & Temperature Sensor (TL)  reference=foundation.enum.MeasurementReference.absolute  pressure=false  pressure_spec=foundation.enum.PressureMeasementSpec.Absolute  temperature=true
      settings: InternalSimscapePortConfiguration="{\"Bottom\":[{\"id\":\"T\",\"label\":\"T\",\"type\":\"output\"}],\"Left\":[{\"id\":\"A\",\"label\":\"A\",\"type\":\"foundation.thermal_liquid.thermal_liquid\"}],\"Right\":[],\"Top\":[]}"
  SMAStage1InletFluidTempPS : nesl_utility/PS-Simulink Converter  PhysicalDomain=network_engine_domain  SubClassName=ps_output  LeftPortType=input  RightPortType=output  PseudoPeriodic=off  Frequencies=[]  VectorFormat=1-D array  Unit=K  AffineConversion=off
  SMAStage1InletFluidTempSensor : fl_lib/Thermal Liquid/Sensors/Pressure & Temperature Sensor (TL)  reference=foundation.enum.MeasurementReference.absolute  pressure=false  pressure_spec=foundation.enum.PressureMeasementSpec.Absolute  temperature=true
      settings: InternalSimscapePortConfiguration="{\"Bottom\":[{\"id\":\"T\",\"label\":\"T\",\"type\":\"output\"}],\"Left\":[{\"id\":\"A\",\"label\":\"A\",\"type\":\"foundation.thermal_liquid.thermal_liquid\"}],\"Right\":[],\"Top\":[]}"
  SMAStage1OutletFluidTempPS : nesl_utility/PS-Simulink Converter  PhysicalDomain=network_engine_domain  SubClassName=ps_output  LeftPortType=input  RightPortType=output  PseudoPeriodic=off  Frequencies=[]  VectorFormat=1-D array  Unit=K  AffineConversion=off
  SMAStage1OutletFluidTempSensor : fl_lib/Thermal Liquid/Sensors/Pressure & Temperature Sensor (TL)  reference=foundation.enum.MeasurementReference.absolute  pressure=false  pressure_spec=foundation.enum.PressureMeasementSpec.Absolute  temperature=true
      settings: InternalSimscapePortConfiguration="{\"Bottom\":[{\"id\":\"T\",\"label\":\"T\",\"type\":\"output\"}],\"Left\":[{\"id\":\"A\",\"label\":\"A\",\"type\":\"foundation.thermal_liquid.thermal_liquid\"}],\"Right\":[],\"Top\":[]}"
  SMAStage1V1PumpSideFluidTempPS : nesl_utility/PS-Simulink Converter  PhysicalDomain=network_engine_domain  SubClassName=ps_output  LeftPortType=input  RightPortType=output  PseudoPeriodic=off  Frequencies=[]  VectorFormat=1-D array  Unit=K  AffineConversion=off
  SMAStage1V1PumpSideFluidTempSensor : fl_lib/Thermal Liquid/Sensors/Pressure & Temperature Sensor (TL)  reference=foundation.enum.MeasurementReference.absolute  pressure=false  pressure_spec=foundation.enum.PressureMeasementSpec.Absolute  temperature=true
      settings: InternalSimscapePortConfiguration="{\"Bottom\":[{\"id\":\"T\",\"label\":\"T\",\"type\":\"output\"}],\"Left\":[{\"id\":\"A\",\"label\":\"A\",\"type\":\"foundation.thermal_liquid.thermal_liquid\"}],\"Right\":[],\"Top\":[]}"
  SMAStage1V1SHEXSideFluidTempPS : nesl_utility/PS-Simulink Converter  PhysicalDomain=network_engine_domain  SubClassName=ps_output  LeftPortType=input  RightPortType=output  PseudoPeriodic=off  Frequencies=[]  VectorFormat=1-D array  Unit=K  AffineConversion=off
  SMAStage1V1SHEXSideFluidTempSensor : fl_lib/Thermal Liquid/Sensors/Pressure & Temperature Sensor (TL)  reference=foundation.enum.MeasurementReference.absolute  pressure=false  pressure_spec=foundation.enum.PressureMeasementSpec.Absolute  temperature=true
      settings: InternalSimscapePortConfiguration="{\"Bottom\":[{\"id\":\"T\",\"label\":\"T\",\"type\":\"output\"}],\"Left\":[{\"id\":\"A\",\"label\":\"A\",\"type\":\"foundation.thermal_liquid.thermal_liquid\"}],\"Right\":[],\"Top\":[]}"
  SMAStage1V5SHEXSideFluidTempPS : nesl_utility/PS-Simulink Converter  PhysicalDomain=network_engine_domain  SubClassName=ps_output  LeftPortType=input  RightPortType=output  PseudoPeriodic=off  Frequencies=[]  VectorFormat=1-D array  Unit=K  AffineConversion=off
  SMAStage1V5SHEXSideFluidTempSensor : fl_lib/Thermal Liquid/Sensors/Pressure & Temperature Sensor (TL)  reference=foundation.enum.MeasurementReference.absolute  pressure=false  pressure_spec=foundation.enum.PressureMeasementSpec.Absolute  temperature=true
      settings: InternalSimscapePortConfiguration="{\"Bottom\":[{\"id\":\"T\",\"label\":\"T\",\"type\":\"output\"}],\"Left\":[{\"id\":\"A\",\"label\":\"A\",\"type\":\"foundation.thermal_liquid.thermal_liquid\"}],\"Right\":[],\"Top\":[]}"
  SMAStage3InletFluidTempPS : nesl_utility/PS-Simulink Converter  PhysicalDomain=network_engine_domain  SubClassName=ps_output  LeftPortType=input  RightPortType=output  PseudoPeriodic=off  Frequencies=[]  VectorFormat=1-D array  Unit=K  AffineConversion=off
  SMAStage3InletFluidTempSensor : fl_lib/Thermal Liquid/Sensors/Pressure & Temperature Sensor (TL)  reference=foundation.enum.MeasurementReference.absolute  pressure=false  pressure_spec=foundation.enum.PressureMeasementSpec.Absolute  temperature=true
      settings: InternalSimscapePortConfiguration="{\"Bottom\":[{\"id\":\"T\",\"label\":\"T\",\"type\":\"output\"}],\"Left\":[{\"id\":\"A\",\"label\":\"A\",\"type\":\"foundation.thermal_liquid.thermal_liquid\"}],\"Right\":[],\"Top\":[]}"
  SMAStage3OutletFluidTempPS : nesl_utility/PS-Simulink Converter  PhysicalDomain=network_engine_domain  SubClassName=ps_output  LeftPortType=input  RightPortType=output  PseudoPeriodic=off  Frequencies=[]  VectorFormat=1-D array  Unit=K  AffineConversion=off
  SMAStage3OutletFluidTempSensor : fl_lib/Thermal Liquid/Sensors/Pressure & Temperature Sensor (TL)  reference=foundation.enum.MeasurementReference.absolute  pressure=false  pressure_spec=foundation.enum.PressureMeasementSpec.Absolute  temperature=true
      settings: InternalSimscapePortConfiguration="{\"Bottom\":[{\"id\":\"T\",\"label\":\"T\",\"type\":\"output\"}],\"Left\":[{\"id\":\"A\",\"label\":\"A\",\"type\":\"foundation.thermal_liquid.thermal_liquid\"}],\"Right\":[],\"Top\":[]}"
  SMAStage3V2HHEXSideFluidTempPS : nesl_utility/PS-Simulink Converter  PhysicalDomain=network_engine_domain  SubClassName=ps_output  LeftPortType=input  RightPortType=output  PseudoPeriodic=off  Frequencies=[]  VectorFormat=1-D array  Unit=K  AffineConversion=off
  SMAStage3V2HHEXSideFluidTempSensor : fl_lib/Thermal Liquid/Sensors/Pressure & Temperature Sensor (TL)  reference=foundation.enum.MeasurementReference.absolute  pressure=false  pressure_spec=foundation.enum.PressureMeasementSpec.Absolute  temperature=true
      settings: InternalSimscapePortConfiguration="{\"Bottom\":[{\"id\":\"T\",\"label\":\"T\",\"type\":\"output\"}],\"Left\":[{\"id\":\"A\",\"label\":\"A\",\"type\":\"foundation.thermal_liquid.thermal_liquid\"}],\"Right\":[],\"Top\":[]}"
  SMAStage3V2PumpSideFluidTempPS : nesl_utility/PS-Simulink Converter  PhysicalDomain=network_engine_domain  SubClassName=ps_output  LeftPortType=input  RightPortType=output  PseudoPeriodic=off  Frequencies=[]  VectorFormat=1-D array  Unit=K  AffineConversion=off
  SMAStage3V2PumpSideFluidTempSensor : fl_lib/Thermal Liquid/Sensors/Pressure & Temperature Sensor (TL)  reference=foundation.enum.MeasurementReference.absolute  pressure=false  pressure_spec=foundation.enum.PressureMeasementSpec.Absolute  temperature=true
      settings: InternalSimscapePortConfiguration="{\"Bottom\":[{\"id\":\"T\",\"label\":\"T\",\"type\":\"output\"}],\"Left\":[{\"id\":\"A\",\"label\":\"A\",\"type\":\"foundation.thermal_liquid.thermal_liquid\"}],\"Right\":[],\"Top\":[]}"
  SMAStage3V6HHEXSideFluidTempPS : nesl_utility/PS-Simulink Converter  PhysicalDomain=network_engine_domain  SubClassName=ps_output  LeftPortType=input  RightPortType=output  PseudoPeriodic=off  Frequencies=[]  VectorFormat=1-D array  Unit=K  AffineConversion=off
  SMAStage3V6HHEXSideFluidTempSensor : fl_lib/Thermal Liquid/Sensors/Pressure & Temperature Sensor (TL)  reference=foundation.enum.MeasurementReference.absolute  pressure=false  pressure_spec=foundation.enum.PressureMeasementSpec.Absolute  temperature=true
      settings: InternalSimscapePortConfiguration="{\"Bottom\":[{\"id\":\"T\",\"label\":\"T\",\"type\":\"output\"}],\"Left\":[{\"id\":\"A\",\"label\":\"A\",\"type\":\"foundation.thermal_liquid.thermal_liquid\"}],\"Right\":[],\"Top\":[]}"
  SMAValveCmdPS{1..6} (6 alike) : nesl_utility/Simulink-PS Converter  PhysicalDomain=network_engine_domain  SubClassName=ps_input  LeftPortType=input  RightPortType=output  PseudoPeriodic=off  Frequencies=[]  NoiseDistribution=none  NoiseParameters=[]  Unit=MPa  AffineConversion=off  FilteringAndDerivatives=provide  SimscapeFilterOrder=1  InputFilterTimeConstant=0.001  UdotUserProvided=0
  SMAValveCommandFromWorkspace : FromWorkspace  VariableName=SMA_L_valve_command  OutputAfterFinalValue=Holding final value
      settings: AttributesFormatString=Four-stage valve command input for route gates
  SMA_Demux : Demux  Outputs=6
      settings: DisplayOption=none
  SMA_PumpInletConnectingPipeVolume : fl_lib/Thermal Liquid/Elements/Constant Volume Chamber (TL)  volume=sma_pump_manifold_volume_m3 m^3  num_ports=foundation.enum.num_ports.two  area_A=sma_connecting_pipe_flow_area_m2 m^2  area_B=sma_connecting_pipe_flow_area_m2 m^2  area_C=0.01 m^2  area_D=0.01 m^2  p_I_specify=on  p_I_priority=Low  p_I=sma_pump_manifold_p_init_MPa MPa  p_I_nominal_specify=off  p_I_nominal_value=1  p_I_nominal_unit=MPa  T_I_specify=on  T_I_priority=Low  T_I=sma_pump_manifold_T_init_K K  T_I_nominal_specify=off  T_I_nominal_value=1  T_I_nominal_unit=K  u_I_specify=off  u_I_priority=None  u_I=83.906 kJ/kg  u_I_nominal_specify=off  u_I_nominal_value=1  u_I_nominal_unit=kJ/kg  rho_I_specify=off  rho_I_priority=None  rho_I=998.21 kg/m^3  rho_I_nominal_specify=off  rho_I_nominal_value=1  rho_I_nominal_unit=kg/m^3
      settings: InternalSimscapePortConfiguration="{\"Bottom\":[],\"Left\":[{\"id\":\"A\",\"label\":\"A\",\"type\":\"foundation.thermal_liquid.thermal_liquid\"},{\"id\":\"H\",\"label\":\"H\",\"type\":\"foundation.thermal.thermal\"}],\"Right\":[{\"id\":\"B\",\"label\":\"B\",\"type\":\"foundation.thermal_liquid.thermal_liquid\"}],\"Top\":[]}"
  SMA_PumpOutletConnectingPipeVolume : fl_lib/Thermal Liquid/Elements/Constant Volume Chamber (TL)  volume=sma_pump_manifold_volume_m3 m^3  num_ports=foundation.enum.num_ports.two  area_A=sma_connecting_pipe_flow_area_m2 m^2  area_B=sma_connecting_pipe_flow_area_m2 m^2  area_C=0.01 m^2  area_D=0.01 m^2  p_I_specify=on  p_I_priority=Low  p_I=sma_pump_manifold_p_init_MPa MPa  p_I_nominal_specify=off  p_I_nominal_value=1  p_I_nominal_unit=MPa  T_I_specify=on  T_I_priority=Low  T_I=sma_pump_manifold_T_init_K K  T_I_nominal_specify=off  T_I_nominal_value=1  T_I_nominal_unit=K  u_I_specify=off  u_I_priority=None  u_I=83.906 kJ/kg  u_I_nominal_specify=off  u_I_nominal_value=1  u_I_nominal_unit=kJ/kg  rho_I_specify=off  rho_I_priority=None  rho_I=998.21 kg/m^3  rho_I_nominal_specify=off  rho_I_nominal_value=1  rho_I_nominal_unit=kg/m^3
      settings: InternalSimscapePortConfiguration="{\"Bottom\":[],\"Left\":[{\"id\":\"A\",\"label\":\"A\",\"type\":\"foundation.thermal_liquid.thermal_liquid\"},{\"id\":\"H\",\"label\":\"H\",\"type\":\"foundation.thermal.thermal\"}],\"Right\":[{\"id\":\"B\",\"label\":\"B\",\"type\":\"foundation.thermal_liquid.thermal_liquid\"}],\"Top\":[]}"
  SMA_ThermalLiquidSettings : fl_lib/Thermal Liquid/Utilities/Thermal Liquid Settings (TL)  table_dimensions=1  T_TLU=[273.16;283.16;293.16;303.16;313.16;323.16;333.16;343.16;353.16;363.16;373.16;383.16;393.16;403.16;413.16] K  p_TLU=[0.01, 0.1, 5 : 5 : 50] MPa  p_atm=0.5 MPa  pT_region_flag=0  T_min=273.16 K  T_max=405 K  p_min=0.01 MPa  p_max=50 MPa  T_min_1D=273.16 K  T_max_1D=413.16 K  p_min_1D=0.45 MPa  p_max_1D=5 MPa  pT_validity_TLU=[1, 1, 1, 1, 1, 1, 1, 1, 1, 1, 1, 1; 1, 1, 1, 1, 1, 1, 1, 1, 1, 1, 1, 1; 1, 1, 1, 1, 1, 1, 1, 1, 1, 1, 1, 1; 1, 1, 1, 1, 1, 1, 1, 1, 1, 1, 1, 1; 1, 1, 1, 1, 1, 1, 1, 1, 1, 1, 1, 1; 0, 1, 1, 1, 1, 1, 1, 1, 1, 1, 1, 1; 0, 1, 1, 1, 1, 1, 1, 1, 1, 1, 1, 1; 0, 1, 1, 1, 1, 1, 1, 1, 1, 1, 1, 1; 0, 1, 1, 1, 1, 1, 1, 1, 1, 1, 1, 1; 0, 1, 1, 1, 1, 1, 1, 1, 1, 1, 1, 1; 0, 0, 1, 1, 1, 1, 1, 1, 1, 1, 1, 1]  properties_range_check=simscape.enum.assert.action.error  rho_parameterization_2D=1  rho_parameterization_1D=1  rho_TLU=[999.7973, 999.8431, 1002.3216, 1004.8218, 1007.293, 1009.7358, 1012.1506, 1014.5379, 1016.8979, 1019.2311, 1021.538, 1023.8188; 999.6579, 999.7009, 1002.0303, 1004.382, 1006.7084, 1009.0101, 1011.2874, 1013.5407, 1015.7703, 1017.9766, 1020.1599, 1022.3206; 998.1632, 998.2045, 1000.4375, 1002.6924, 1004.9239, 1007.1324, 1009.3183, 1011.4819, 1013.6236, 1015.7438, 1017.8428, 1019.921; 995.6057, 995.6458, 997.81864, 1000.0128, 1002.1841, 1004.3332, 1006.4603, 1008.566, 1010.6505, 1012.7144, 1014.758, 1016.7815; 992.1724, 992.2119, 994.35133, 996.5113, 998.6484, 1000.7633, 1002.8563, 1004.928, 1006.9788, 1009.009, 1011.0192, 1013.0097; 988.02, 988.0299, 990.15684, 992.3035, 994.4268, 996.5273, 998.6056, 1000.6622, 1002.6976, 1004.7123, 1006.7067, 1008.6813; 983.18, 983.1901, 985.3217, 987.4721, 989.5983, 991.7008, 993.7803, 995.8374, 997.8726, 999.8864, 1001.8795, 1003.8522; 977.75, 977.7583, 979.9094, 982.0783, 984.2216, 986.34, 988.4343, 990.505, 992.5529, 994.5786, 996.5825, 998.5654; 971.77, 971.7836, 973.96734, 976.1678, 978.3409, 980.4876, 982.6087, 984.7049, 986.7768, 988.8254, 990.8511, 992.8545; 965.26, 965.3023, 967.53107, 969.7753, 971.9901, 974.1764, 976.3354, 978.4676, 980.5741, 982.6556, 984.7129, 986.7465; 958.62, 958.6315, 960.627, 962.9267, 965.1944, 967.4314, 969.6387, 971.8173, 973.9681, 976.0921, 978.19, 980.2628] kg/m^3  beta_TLU=[1.9649, 1.9654, 1.9929, 2.0213, 2.0499, 2.0787, 2.1078, 2.1372, 2.1668, 2.1966, 2.2268, 2.2572; 2.0913, 2.0918, 2.1191, 2.1471, 2.1752, 2.2036, 2.2322, 2.261, 2.2899, 2.3191, 2.3485, 2.3781; 2.1786, 2.1791, 2.2067, 2.235, 2.2634, 2.2919, 2.3206, 2.3494, 2.3784, 2.4075, 2.4367, 2.4661; 2.2332, 2.2337, 2.2619, 2.2908, 2.3197, 2.3487, 2.3778, 2.407, 2.4363, 2.4657, 2.4951, 2.5246; 2.26, 2.2605, 2.2895, 2.3191, 2.3487, 2.3784, 2.4081, 2.4378, 2.4675, 2.4973, 2.5272, 2.5571; 2.2638, 2.2638, 2.2936, 2.324, 2.3544, 2.3848, 2.4151, 2.4455, 2.4758, 2.5062, 2.5365, 2.5669; 2.2472, 2.2472, 2.2779, 2.3092, 2.3403, 2.3715, 2.4025, 2.4336, 2.4646, 2.4955, 2.5264, 2.5573; 2.214, 2.214, 2.2455, 2.2776, 2.3096, 2.3415, 2.3733, 2.405, 2.4367, 2.4683, 2.4998, 2.5313; 2.1668, 2.1668, 2.1992, 2.2321, 2.2649, 2.2976, 2.3301, 2.3626, 2.3949, 2.4272, 2.4593, 2.4914; 2.1081, 2.1081, 2.1413, 2.175, 2.2086, 2.2421, 2.2754, 2.3085, 2.3415, 2.3744, 2.4072, 2.4399; 2.0494, 2.0494, 2.0739, 2.1084, 2.1428, 2.177, 2.211, 2.2449, 2.2786, 2.3121, 2.3455, 2.3788] GPa  alpha_TLU=1e-4 * [-.679, -.676, -.49, -.307, -.13, .041, .206, .365, .519, .668, .811, .949; .878, .881, .998, 1.114, 1.227, 1.337, 1.445, 1.549, 1.651, 1.75, 1.846, 1.939; 2.068, 2.069, 2.141, 2.213, 2.283, 2.352, 2.42, 2.486, 2.551, 2.614, 2.676, 2.736; 3.034, 3.035, 3.074, 3.113, 3.152, 3.191, 3.229, 3.267, 3.305, 3.341, 3.377, 3.413; 3.855, 3.856, 3.87, 3.884, 3.899, 3.914, 3.93, 3.946, 3.961, 3.977, 3.993, 4.009; 4.578, 4.578, 4.572, 4.566, 4.562, 4.558, 4.555, 4.552, 4.55, 4.549, 4.548, 4.547; 5.233, 5.233, 5.209, 5.186, 5.165, 5.144, 5.125, 5.107, 5.09, 5.074, 5.059, 5.045; 5.84, 5.84, 5.801, 5.762, 5.725, 5.691, 5.657, 5.625, 5.595, 5.566, 5.538, 5.512; 6.414, 6.414, 6.36, 6.307, 6.256, 6.208, 6.161, 6.117, 6.074, 6.033, 5.994, 5.956; 6.967, 6.967, 6.898, 6.831, 6.766, 6.705, 6.646, 6.589, 6.535, 6.482, 6.432, 6.384; 7.519, 7.519, 7.423, 7.342, 7.264, 7.189, 7.118, 7.049, 6.983, 6.92, 6.859, 6.8] 1/K  rho_TLU_2=[999.7973, 999.8431, 1002.3216, 1004.8218, 1007.293, 1009.7358, 1012.1506, 1014.5379, 1016.8979, 1019.2311, 1021.538, 1023.8188; 999.6579, 999.7009, 1002.0303, 1004.382, 1006.7084, 1009.0101, 1011.2874, 1013.5407, 1015.7703, 1017.9766, 1020.1599, 1022.3206; 998.1632, 998.2045, 1000.4375, 1002.6924, 1004.9239, 1007.1324, 1009.3183, 1011.4819, 1013.6236, 1015.7438, 1017.8428, 1019.921; 995.6057, 995.6458, 997.81864, 1000.0128, 1002.1841, 1004.3332, 1006.4603, 1008.566, 1010.6505, 1012.7144, 1014.758, 1016.7815; 992.1724, 992.2119, 994.35133, 996.5113, 998.6484, 1000.7633, 1002.8563, 1004.928, 1006.9788, 1009.009, 1011.0192, 1013.0097; 988.02, 988.0299, 990.15684, 992.3035, 994.4268, 996.5273, 998.6056, 1000.6622, 1002.6976, 1004.7123, 1006.7067, 1008.6813; 983.18, 983.1901, 985.3217, 987.4721, 989.5983, 991.7008, 993.7803, 995.8374, 997.8726, 999.8864, 1001.8795, 1003.8522; 977.75, 977.7583, 979.9094, 982.0783, 984.2216, 986.34, 988.4343, 990.505, 992.5529, 994.5786, 996.5825, 998.5654; 971.77, 971.7836, 973.96734, 976.1678, 978.3409, 980.4876, 982.6087, 984.7049, 986.7768, 988.8254, 990.8511, 992.8545; 965.26, 965.3023, 967.53107, 969.7753, 971.9901, 974.1764, 976.3354, 978.4676, 980.5741, 982.6556, 984.7129, 986.7465; 958.62, 958.6315, 960.627, 962.9267, 965.1944, 967.4314, 969.6387, 971.8173, 973.9681, 976.0921, 978.19, 980.2628] kg/m^3  rho_ref_3=998.21 kg/m^3  T_ref_3=293.16 K  p_ref_3=0.101325 MPa  beta_const_3=2.1791 GPa  alpha_const_3=2.0691e-4 1/K  rho_TLU_4=[1000.047692;999.8910379;998.3863142;995.8262391;992.3948132;988.216282;983.3792011;977.9489783;971.9748358;965.4939159;958.5338333;951.1143215;943.2483073;934.9425941;926.1982521] kg/m^3  beta_const_4=2.15 GPa  p_ref_4=0.5 MPa  rho_ref_5=998.21 kg/m^3  T_ref_5=293.16 K  p_ref_5=0.101325 MPa  beta_const_5=2.1791 GPa  alpha_const_5=2.0691e-4 1/K  u_parameterization_2D=1  u_parameterization_1D=1  u_TLU=[.0002, .0018, .086, .1588, .219, .267, .3034, .3288, .3436, .3483, .3435, .3294; 42.062, 42.06, 41.935, 41.804, 41.668, 41.527, 41.382, 41.233, 41.081, 40.924, 40.763, 40.599; 83.953, 83.948, 83.651, 83.349, 83.049, 82.749, 82.451, 82.153, 81.856, 81.56, 81.265, 80.971; 125.77, 125.76, 125.31, 124.86, 124.41, 123.97, 123.53, 123.1, 122.68, 122.25, 121.84, 121.42; 167.57, 167.56, 166.96, 166.37, 165.79, 165.21, 164.65, 164.09, 163.54, 163, 162.46, 161.94; 209.36, 209.36, 208.63, 207.9, 207.19, 206.48, 205.79, 205.11, 204.45, 203.79, 203.14, 202.5; 251.19, 251.19, 250.33, 249.47, 248.62, 247.79, 246.98, 246.18, 245.39, 244.62, 243.86, 243.12; 293.06, 293.06, 292.07, 291.07, 290.1, 289.14, 288.2, 287.28, 286.38, 285.49, 284.62, 283.77; 334.99, 334.99, 333.86, 332.73, 331.63, 330.54, 329.48, 328.44, 327.41, 326.41, 325.43, 324.46; 377, 377, 375.73, 374.46, 373.22, 372, 370.81, 369.64, 368.5, 367.38, 366.27, 365.19; 419.01, 419.01, 417.69, 416.27, 414.89, 413.54, 412.21, 410.91, 409.64, 408.4, 407.17, 405.98] kJ/kg  cp_TLU=[4.2199, 4.2194, 4.1957, 4.1726, 4.1508, 4.13, 4.1103, 4.0916, 4.0738, 4.0569, 4.0408, 4.0254; 4.1955, 4.1951, 4.1769, 4.1592, 4.1422, 4.1259, 4.1103, 4.0954, 4.0812, 4.0676, 4.0545, 4.0421; 4.1843, 4.184, 4.169, 4.1543, 4.1401, 4.1264, 4.1133, 4.1007, 4.0885, 4.0768, 4.0656, 4.0548; 4.1801, 4.1798, 4.1667, 4.1538, 4.1413, 4.1293, 4.1177, 4.1064, 4.0956, 4.0851, 4.075, 4.0653; 4.1796, 4.1794, 4.1675, 4.1558, 4.1444, 4.1334, 4.1227, 4.1123, 4.1023, 4.0926, 4.0832, 4.0741; 4.1813, 4.1813, 4.1702, 4.1592, 4.1484, 4.138, 4.1279, 4.1181, 4.1086, 4.0993, 4.0903, 4.0816; 4.185, 4.185, 4.1742, 4.1636, 4.1532, 4.1432, 4.1334, 4.1239, 4.1146, 4.1056, 4.0969, 4.0884; 4.1901, 4.1901, 4.1795, 4.169, 4.1588, 4.1489, 4.1393, 4.1299, 4.1207, 4.1118, 4.1032, 4.0947; 4.1968, 4.1968, 4.1862, 4.1757, 4.1655, 4.1555, 4.1458, 4.1364, 4.1273, 4.1183, 4.1096, 4.1012; 4.2052, 4.2052, 4.1944, 4.1837, 4.1733, 4.1632, 4.1534, 4.1438, 4.1345, 4.1255, 4.1166, 4.108; 4.2136, 4.2136, 4.2045, 4.1935, 4.1828, 4.1724, 4.1623, 4.1524, 4.1429, 4.1335, 4.1245, 4.1157] kJ/kg/K  u_TLU_2=[.0002, .0018, .086, .1588, .219, .267, .3034, .3288, .3436, .3483, .3435, .3294; 42.062, 42.06, 41.935, 41.804, 41.668, 41.527, 41.382, 41.233, 41.081, 40.924, 40.763, 40.599; 83.953, 83.948, 83.651, 83.349, 83.049, 82.749, 82.451, 82.153, 81.856, 81.56, 81.265, 80.971; 125.77, 125.76, 125.31, 124.86, 124.41, 123.97, 123.53, 123.1, 122.68, 122.25, 121.84, 121.42; 167.57, 167.56, 166.96, 166.37, 165.79, 165.21, 164.65, 164.09, 163.54, 163, 162.46, 161.94; 209.36, 209.36, 208.63, 207.9, 207.19, 206.48, 205.79, 205.11, 204.45, 203.79, 203.14, 202.5; 251.19, 251.19, 250.33, 249.47, 248.62, 247.79, 246.98, 246.18, 245.39, 244.62, 243.86, 243.12; 293.06, 293.06, 292.07, 291.07, 290.1, 289.14, 288.2, 287.28, 286.38, 285.49, 284.62, 283.77; 334.99, 334.99, 333.86, 332.73, 331.63, 330.54, 329.48, 328.44, 327.41, 326.41, 325.43, 324.46; 377, 377, 375.73, 374.46, 373.22, 372, 370.81, 369.64, 368.5, 367.38, 366.27, 365.19; 419.01, 419.01, 417.69, 416.27, 414.89, 413.54, 412.21, 410.91, 409.64, 408.4, 407.17, 405.98] kJ/kg  cp_TLU_3=[4.2199, 4.2194, 4.1957, 4.1726, 4.1508, 4.13, 4.1103, 4.0916, 4.0738, 4.0569, 4.0408, 4.0254; 4.1955, 4.1951, 4.1769, 4.1592, 4.1422, 4.1259, 4.1103, 4.0954, 4.0812, 4.0676, 4.0545, 4.0421; 4.1843, 4.184, 4.169, 4.1543, 4.1401, 4.1264, 4.1133, 4.1007, 4.0885, 4.0768, 4.0656, 4.0548; 4.1801, 4.1798, 4.1667, 4.1538, 4.1413, 4.1293, 4.1177, 4.1064, 4.0956, 4.0851, 4.075, 4.0653; 4.1796, 4.1794, 4.1675, 4.1558, 4.1444, 4.1334, 4.1227, 4.1123, 4.1023, 4.0926, 4.0832, 4.0741; 4.1813, 4.1813, 4.1702, 4.1592, 4.1484, 4.138, 4.1279, 4.1181, 4.1086, 4.0993, 4.0903, 4.0816; 4.185, 4.185, 4.1742, 4.1636, 4.1532, 4.1432, 4.1334, 4.1239, 4.1146, 4.1056, 4.0969, 4.0884; 4.1901, 4.1901, 4.1795, 4.169, 4.1588, 4.1489, 4.1393, 4.1299, 4.1207, 4.1118, 4.1032, 4.0947; 4.1968, 4.1968, 4.1862, 4.1757, 4.1655, 4.1555, 4.1458, 4.1364, 4.1273, 4.1183, 4.1096, 4.1012; 4.2052, 4.2052, 4.1944, 4.1837, 4.1733, 4.1632, 4.1534, 4.1438, 4.1345, 4.1255, 4.1166, 4.108; 4.2136, 4.2136, 4.2045, 4.1935, 4.1828, 4.1724, 4.1623, 4.1524, 4.1429, 4.1335, 4.1245, 4.1157] kJ/kg/K  u_TLU_4=[0.009195591107;42.04935692;83.92921694;125.7370066;167.5155824;209.2925951;251.0909039;292.9318876;334.8364138;376.8251884;418.9190578;461.1394123;503.5087057;546.0510694;588.793005] kJ/kg  cp_TLU_5=[4.2199; 4.1955; 4.1843; 4.1801; 4.1796; 4.1813; 4.185; 4.1901; 4.1968; 4.2052; 4.2136] kJ/kg/K  nu_TLU=[1.7917, 1.7914, 1.7763, 1.7615, 1.7473, 1.7338, 1.7208, 1.7085, 1.6967, 1.6854, 1.6747, 1.6645; 1.3061, 1.3059, 1.2986, 1.2914, 1.2845, 1.2779, 1.2716, 1.2656, 1.2598, 1.2543, 1.2491, 1.2441; 1.0032, 1.0032, .9995, .9959, .9924, .9891, .9859, .9829, .9801, .9774, .9748, .9724; .8006, .8005, .7987, .797, .7953, .7937, .7922, .7908, .7894, .7881, .787, .7859; .6577, .6577, .657, .6562, .6555, .6548, .6543, .6537, .6532, .6528, .6523, .652; .553, .553, .5529, .5527, .5526, .5525, .5524, .5524, .5524, .5524, .5524, .5525; .4739, .4739, .4741, .4743, .4745, .4747, .475, .4753, .4755, .4758, .4762, .4765; .4127, .4127, .4131, .4135, .4139, .4143, .4148, .4152, .4157, .4162, .4167, .4172; .3643, .3643, .3648, .3654, .3659, .3665, .367, .3676, .3682, .3688, .3694, .37; .3254, .3254, .3261, .3267, .3273, .328, .3286, .3293, .3299, .3306, .3312, .3319; .2866, .2866, .2945, .2952, .2959, .2965, .2972, .2979, .2986, .2993, .3, .3007] mm^2/s  nu_TLU_2=[1.790149606;1.305308358;1.002847726;0.8003847494;0.6576599304;0.5530269976;0.4739457078;0.4127054691;0.3643312332;0.3254838619;0.2938478789;0.2677732136;0.246056468;0.227802409;0.2123334626] mm^2/s  k_TLU=[561.04, 561.09, 563.8, 566.56, 569.32, 572.08, 574.82, 577.54, 580.24, 582.92, 585.57, 588.18; 580.02, 580.07, 582.45, 584.88, 587.32, 589.75, 592.18, 594.61, 597.02, 599.42, 601.8, 604.16; 598.44, 598.48, 600.73, 603.03, 605.33, 607.64, 609.94, 612.24, 614.54, 616.82, 619.1, 621.36; 615.48, 615.52, 617.73, 620, 622.26, 624.54, 626.81, 629.07, 631.34, 633.6, 635.85, 638.09; 630.6, 630.64, 632.87, 635.15, 637.44, 639.72, 642.01, 644.29, 646.57, 648.84, 651.11, 653.36; 643.61, 643.61, 645.88, 648.21, 650.53, 652.86, 655.18, 657.51, 659.82, 662.14, 664.44, 666.74; 654.39, 654.39, 656.73, 659.12, 661.5, 663.89, 666.27, 668.65, 671.02, 673.38, 675.74, 678.09; 663.13, 663.13, 665.54, 668, 670.46, 672.91, 675.36, 677.8, 680.24, 682.67, 685.09, 687.5; 670.02, 670.02, 672.51, 675.05, 677.59, 680.12, 682.64, 685.16, 687.67, 690.17, 692.66, 695.14; 675.27, 675.27, 677.85, 680.48, 683.11, 685.73, 688.34, 690.94, 693.53, 696.11, 698.68, 701.24; 680.52, 680.52, 681.77, 684.5, 687.22, 689.94, 692.64, 695.34, 698.02, 700.69, 703.35, 706] mW/m/K  k_TLU_2=[555.9805115;579.057427;598.2630374;614.6297471;628.7193807;640.8549223;651.2352248;659.9939082;667.2300958;673.0243742;677.4468439;680.5609271;682.4249382;683.0925227;682.612562] mW/m/K
  SMA_V1_SHEX_to_pump : SimscapeFluids_lib/Thermal Liquid/Valves & Orifices/Flow Coefficient Parameterized Valve (TL)  flow_coeff_spec=fluids.thermal_liquid.valves.enum.flow_coeff_spec.cv  Cv_max=1  Cv_min=sma_source_select_valve_min_Cv  Kv_max=1  Kv_min=sma_source_select_valve_min_Cv  valve_character=fluids.thermal_liquid.valves.enum.valve_opening_spec.linear  rangeability=50  alpha=2  area=sma_pipe_fa m^2  Re_c=150  smoothing_factor=0.01
      settings: AttributesFormatString=Retained mature route gate V1  InternalSimscapePortConfiguration="{\"Bottom\":[],\"Left\":[{\"id\":\"A\",\"label\":\"A\",\"type\":\"foundation.thermal_liquid.thermal_liquid\"},{\"id\":\"L\",\"label\":\"L\",\"type\":\"input\"}],\"Right\":[{\"id\":\"B\",\"label\":\"B\",\"type\":\"foundation.thermal_liquid.thermal_liquid\"}],\"Top\":[]}"
  SMA_V2_HHEX_to_pump : SimscapeFluids_lib/Thermal Liquid/Valves & Orifices/Flow Coefficient Parameterized Valve (TL)  flow_coeff_spec=fluids.thermal_liquid.valves.enum.flow_coeff_spec.cv  Cv_max=1  Cv_min=sma_source_select_valve_min_Cv  Kv_max=1  Kv_min=sma_source_select_valve_min_Cv  valve_character=fluids.thermal_liquid.valves.enum.valve_opening_spec.linear  rangeability=50  alpha=2  area=sma_pipe_fa m^2  Re_c=150  smoothing_factor=0.01
      settings: AttributesFormatString=Retained mature route gate V1  InternalSimscapePortConfiguration="{\"Bottom\":[],\"Left\":[{\"id\":\"A\",\"label\":\"A\",\"type\":\"foundation.thermal_liquid.thermal_liquid\"},{\"id\":\"L\",\"label\":\"L\",\"type\":\"input\"}],\"Right\":[{\"id\":\"B\",\"label\":\"B\",\"type\":\"foundation.thermal_liquid.thermal_liquid\"}],\"Top\":[]}"
  SMA_V3_pump_to_heat_path : SimscapeFluids_lib/Thermal Liquid/Valves & Orifices/Flow Coefficient Parameterized Valve (TL)  flow_coeff_spec=fluids.thermal_liquid.valves.enum.flow_coeff_spec.cv  Cv_max=1  Cv_min=sma_route_valve_min_Cv  Kv_max=1  Kv_min=sma_route_valve_min_Cv  valve_character=fluids.thermal_liquid.valves.enum.valve_opening_spec.linear  rangeability=50  alpha=2  area=sma_pipe_fa m^2  Re_c=150  smoothing_factor=0.01
      settings: AttributesFormatString=Retained mature route gate V1  InternalSimscapePortConfiguration="{\"Bottom\":[],\"Left\":[{\"id\":\"A\",\"label\":\"A\",\"type\":\"foundation.thermal_liquid.thermal_liquid\"},{\"id\":\"L\",\"label\":\"L\",\"type\":\"input\"}],\"Right\":[{\"id\":\"B\",\"label\":\"B\",\"type\":\"foundation.thermal_liquid.thermal_liquid\"}],\"Top\":[]}"
  SMA_V4_pump_to_cool_path : SimscapeFluids_lib/Thermal Liquid/Valves & Orifices/Flow Coefficient Parameterized Valve (TL)  flow_coeff_spec=fluids.thermal_liquid.valves.enum.flow_coeff_spec.cv  Cv_max=1  Cv_min=sma_route_valve_min_Cv  Kv_max=1  Kv_min=sma_route_valve_min_Cv  valve_character=fluids.thermal_liquid.valves.enum.valve_opening_spec.linear  rangeability=50  alpha=2  area=sma_pipe_fa m^2  Re_c=150  smoothing_factor=0.01
      settings: AttributesFormatString=Retained mature route gate V1  InternalSimscapePortConfiguration="{\"Bottom\":[],\"Left\":[{\"id\":\"A\",\"label\":\"A\",\"type\":\"foundation.thermal_liquid.thermal_liquid\"},{\"id\":\"L\",\"label\":\"L\",\"type\":\"input\"}],\"Right\":[{\"id\":\"B\",\"label\":\"B\",\"type\":\"foundation.thermal_liquid.thermal_liquid\"}],\"Top\":[]}"
  SMA_V5_SMA_to_SHEX : SimscapeFluids_lib/Thermal Liquid/Valves & Orifices/Flow Coefficient Parameterized Valve (TL)  flow_coeff_spec=fluids.thermal_liquid.valves.enum.flow_coeff_spec.cv  Cv_max=1  Cv_min=sma_route_valve_min_Cv  Kv_max=1  Kv_min=sma_route_valve_min_Cv  valve_character=fluids.thermal_liquid.valves.enum.valve_opening_spec.linear  rangeability=50  alpha=2  area=sma_pipe_fa m^2  Re_c=150  smoothing_factor=0.01
      settings: AttributesFormatString=Retained mature route gate V1  InternalSimscapePortConfiguration="{\"Bottom\":[],\"Left\":[{\"id\":\"A\",\"label\":\"A\",\"type\":\"foundation.thermal_liquid.thermal_liquid\"},{\"id\":\"L\",\"label\":\"L\",\"type\":\"input\"}],\"Right\":[{\"id\":\"B\",\"label\":\"B\",\"type\":\"foundation.thermal_liquid.thermal_liquid\"}],\"Top\":[]}"
  SMA_V6_SMA_to_HHEX : SimscapeFluids_lib/Thermal Liquid/Valves & Orifices/Flow Coefficient Parameterized Valve (TL)  flow_coeff_spec=fluids.thermal_liquid.valves.enum.flow_coeff_spec.cv  Cv_max=1  Cv_min=sma_route_valve_min_Cv  Kv_max=1  Kv_min=sma_route_valve_min_Cv  valve_character=fluids.thermal_liquid.valves.enum.valve_opening_spec.linear  rangeability=50  alpha=2  area=sma_pipe_fa m^2  Re_c=150  smoothing_factor=0.01
      settings: AttributesFormatString=Retained mature route gate V1  InternalSimscapePortConfiguration="{\"Bottom\":[],\"Left\":[{\"id\":\"A\",\"label\":\"A\",\"type\":\"foundation.thermal_liquid.thermal_liquid\"},{\"id\":\"L\",\"label\":\"L\",\"type\":\"input\"}],\"Right\":[{\"id\":\"B\",\"label\":\"B\",\"type\":\"foundation.thermal_liquid.thermal_liquid\"}],\"Top\":[]}"
  Scope : Scope  Commented=on
      settings: ActiveDisplayYMinimum=285.06328  ActiveDisplayYMaximum=299.6041  DataLoggingVariableName=Tin
  Scope1 : Scope  Commented=on
      settings: ActiveDisplayYMinimum=298.12503  ActiveDisplayYMaximum=298.37477  DataLoggingVariableName=Tout
  Simulink-PS Converter{,1..5} (6 alike) : nesl_utility/Simulink-PS Converter  PhysicalDomain=network_engine_domain  SubClassName=ps_input  LeftPortType=input  RightPortType=output  PseudoPeriodic=off  Frequencies=[]  NoiseDistribution=none  NoiseParameters=[]  Unit=1  AffineConversion=off  FilteringAndDerivatives=provide  SimscapeFilterOrder=1  InputFilterTimeConstant=0.001  UdotUserProvided=0
  Solver Configuration : nesl_utility/Solver Configuration  PhysicalDomain=network_engine_domain  SubClassName=solver  LeftPortType=input  RightPortType=generic  Tones=[]  Harmonics=[]  SimulateNoise=off  Profile=off  UseLocalSampling=off  EnableSwitchedLinearOptims=on  FrequencyDomain=off  UseCCode=off  RelTol=0.001  AbsTol=1e-06  MinStep=1e-09  ToWorkspace=off  RevertToSquareIcSolve=off  NumHomotopyIterations=100  PhasorMode=off  PhasorModeNumHarmonics=1  ConsistencySolver=NEWTON_FTOL  IndexReductionMethod=DerivativeReplacement  DoDC=off  ResidualTolerance=0.001  ConsistencyTolSource=GLOBAL  ConsistencyAbsTol=0.001  ConsistencyRelTol=0.001  ConsistencyTolFactor=0.001  UseLocalSolver=on  LocalSolverChoice=NE_BACKWARD_EULER_ADVANCER  ResolveIndetEquations=on  FunctionEvalNumThread=1  LocalSolverSampleTime=0.001  DoFixedCost=off  MaxNonlinIter=3  MaxModeIter=2  ComputeImpulses=off  ImpulseIterations=2  LinearAlgebra=auto  LinearAlgebraNumThread=0  EquationFormulation=NE_TIME_EF  DelaysMemoryBudget=1024  AutomaticFiltering=on  FilteringTimeConstant=0.001  PartitionStorageMethod=AS_NEEDED  PartitionMemoryBudget=1024  PartitionMethod=FAST  MultibodyUseLocalSolver=off  MultibodyLocalSolverChoice=ODE1  MultibodyLocalSolverSampleTime=0.001
  ToWorkspace_ECC_Constitutive21_Output : ToWorkspace  VariableName=ECC_constitutive21_output  SaveFormat=Structure With Time  SampleTime=-1
  ToWorkspace_ECC_Q_SE_constitutive_W : ToWorkspace  VariableName=ECC_Q_SE_constitutive_W  SaveFormat=Structure With Time  SampleTime=-1
  ToWorkspace_ECC_Q_SMA_constitutive_W : ToWorkspace  VariableName=ECC_Q_SMA_constitutive_W  SaveFormat=Structure With Time  SampleTime=-1
  ToWorkspace_cold_buffer_temp_out : ToWorkspace  VariableName=cold_buffer_temp_out  SaveFormat=Structure With Time  SampleTime=-1
  ToWorkspace_hot_buffer_temp_out : ToWorkspace  VariableName=hot_buffer_temp_out  SaveFormat=Structure With Time  SampleTime=-1
  ToWorkspace_mass_flow_sma_stage13_kgps : ToWorkspace  VariableName=mass_flow_sma_stage13_kgps  SaveFormat=Structure With Time  SampleTime=-1
  ToWorkspace_mass_flow_sma_stage1_route_kgps : ToWorkspace  VariableName=mass_flow_sma_stage1_route_kgps  SaveFormat=Structure With Time  SampleTime=-1
  ToWorkspace_mass_flow_sma_stage3_route_kgps : ToWorkspace  VariableName=mass_flow_sma_stage3_route_kgps  SaveFormat=Structure With Time  SampleTime=-1
  ToWorkspace_mass_flow_v1_cold_inlet_kgps : ToWorkspace  VariableName=mass_flow_v1_cold_inlet_kgps  SaveFormat=Structure With Time  SampleTime=-1
  ToWorkspace_mass_flow_v3_sma_to_hot_kgps : ToWorkspace  VariableName=mass_flow_v3_sma_to_hot_kgps  SaveFormat=Structure With Time  SampleTime=-1
  ToWorkspace_mass_flow_v4_hot_inlet_kgps : ToWorkspace  VariableName=mass_flow_v4_hot_inlet_kgps  SaveFormat=Structure With Time  SampleTime=-1
  ToWorkspace_mass_flow_v6_sma_to_chip_cold_kgps : ToWorkspace  VariableName=mass_flow_v6_sma_to_chip_cold_kgps  SaveFormat=Structure With Time  SampleTime=-1
  ToWorkspace_pressure_command_se_MPa : ToWorkspace  VariableName=pressure_command_se_MPa  SaveFormat=Structure With Time  SampleTime=-1
  ToWorkspace_pressure_command_sma_MPa : ToWorkspace  VariableName=pressure_command_sma_MPa  SaveFormat=Structure With Time  SampleTime=-1
  ToWorkspace_probe_root_cold_buffer_fluid_T_K : ToWorkspace  VariableName=probe_root_cold_buffer_fluid_T_K  SaveFormat=Structure With Time  SampleTime=-1
  ToWorkspace_probe_root_hot_buffer_fluid_T_K : ToWorkspace  VariableName=probe_root_hot_buffer_fluid_T_K  SaveFormat=Structure With Time  SampleTime=-1
  ToWorkspace_probe_root_shex_buffer_fluid_T_K : ToWorkspace  VariableName=probe_root_shex_buffer_fluid_T_K  SaveFormat=Structure With Time  SampleTime=-1
  ToWorkspace_probe_sma_stage13_pump_outlet_T_K : ToWorkspace  VariableName=probe_sma_stage13_pump_outlet_T_K  SaveFormat=Structure With Time  SampleTime=-1
  ToWorkspace_probe_sma_stage1_port1_v3_side_T_K : ToWorkspace  VariableName=probe_sma_stage1_port1_v3_side_T_K  SaveFormat=Structure With Time  SampleTime=-1
  ToWorkspace_probe_sma_stage1_port2_v5_side_T_K : ToWorkspace  VariableName=probe_sma_stage1_port2_v5_side_T_K  SaveFormat=Structure With Time  SampleTime=-1
  ToWorkspace_probe_sma_stage1_v1_pump_side_T_K : ToWorkspace  VariableName=probe_sma_stage1_v1_pump_side_T_K  SaveFormat=Structure With Time  SampleTime=-1
  ToWorkspace_probe_sma_stage1_v1_shex_side_T_K : ToWorkspace  VariableName=probe_sma_stage1_v1_shex_side_T_K  SaveFormat=Structure With Time  SampleTime=-1
  ToWorkspace_probe_sma_stage1_v5_shex_side_T_K : ToWorkspace  VariableName=probe_sma_stage1_v5_shex_side_T_K  SaveFormat=Structure With Time  SampleTime=-1
  ToWorkspace_probe_sma_stage2_port1_v1_side_T_K : ToWorkspace  VariableName=probe_sma_stage2_port1_v1_side_T_K  SaveFormat=Structure With Time  SampleTime=-1
  ToWorkspace_probe_sma_stage2_port2_v3_side_T_K : ToWorkspace  VariableName=probe_sma_stage2_port2_v3_side_T_K  SaveFormat=Structure With Time  SampleTime=-1
  ToWorkspace_probe_sma_stage3_port3_v4_side_T_K : ToWorkspace  VariableName=probe_sma_stage3_port3_v4_side_T_K  SaveFormat=Structure With Time  SampleTime=-1
  ToWorkspace_probe_sma_stage3_port4_v6_side_T_K : ToWorkspace  VariableName=probe_sma_stage3_port4_v6_side_T_K  SaveFormat=Structure With Time  SampleTime=-1
  ToWorkspace_probe_sma_stage3_v2_hhex_side_T_K : ToWorkspace  VariableName=probe_sma_stage3_v2_hhex_side_T_K  SaveFormat=Structure With Time  SampleTime=-1
  ToWorkspace_probe_sma_stage3_v2_pump_side_T_K : ToWorkspace  VariableName=probe_sma_stage3_v2_pump_side_T_K  SaveFormat=Structure With Time  SampleTime=-1
  ToWorkspace_probe_sma_stage3_v6_hhex_side_T_K : ToWorkspace  VariableName=probe_sma_stage3_v6_hhex_side_T_K  SaveFormat=Structure With Time  SampleTime=-1
  ToWorkspace_probe_sma_stage4_port3_v4_side_T_K : ToWorkspace  VariableName=probe_sma_stage4_port3_v4_side_T_K  SaveFormat=Structure With Time  SampleTime=-1
  ToWorkspace_probe_sma_stage4_port4_v6_side_T_K : ToWorkspace  VariableName=probe_sma_stage4_port4_v6_side_T_K  SaveFormat=Structure With Time  SampleTime=-1
  ToWorkspace_probe_v1_cold_inlet_cold_buffer_side_T_K : ToWorkspace  VariableName=probe_v1_cold_inlet_cold_buffer_side_T_K  SaveFormat=Structure With Time  SampleTime=-1
  ToWorkspace_probe_v1_cold_inlet_sma_side_T_K : ToWorkspace  VariableName=probe_v1_cold_inlet_sma_side_T_K  SaveFormat=Structure With Time  SampleTime=-1
  ToWorkspace_probe_v3_sma_to_hot_hot_hx_side_T_K : ToWorkspace  VariableName=probe_v3_sma_to_hot_hot_hx_side_T_K  SaveFormat=Structure With Time  SampleTime=-1
  ToWorkspace_probe_v3_sma_to_hot_sma_side_T_K : ToWorkspace  VariableName=probe_v3_sma_to_hot_sma_side_T_K  SaveFormat=Structure With Time  SampleTime=-1
  ToWorkspace_probe_v4_hot_inlet_hot_buffer_side_T_K : ToWorkspace  VariableName=probe_v4_hot_inlet_hot_buffer_side_T_K  SaveFormat=Structure With Time  SampleTime=-1
  ToWorkspace_probe_v4_hot_inlet_sma_side_T_K : ToWorkspace  VariableName=probe_v4_hot_inlet_sma_side_T_K  SaveFormat=Structure With Time  SampleTime=-1
  ToWorkspace_probe_v6_sma_to_chip_chip_side_T_K : ToWorkspace  VariableName=probe_v6_sma_to_chip_chip_side_T_K  SaveFormat=Structure With Time  SampleTime=-1
  ToWorkspace_probe_v6_sma_to_chip_sma_side_T_K : ToWorkspace  VariableName=probe_v6_sma_to_chip_sma_side_T_K  SaveFormat=Structure With Time  SampleTime=-1
  ToWorkspace_se_cooldown_inlet_fluid_temp_out : ToWorkspace  VariableName=se_cooldown_inlet_fluid_temp_out  SaveFormat=Structure With Time  SampleTime=-1
  ToWorkspace_se_cooldown_outlet_fluid_temp_out : ToWorkspace  VariableName=se_cooldown_outlet_fluid_temp_out  SaveFormat=Structure With Time  SampleTime=-1
  ToWorkspace_se_hold_inlet_fluid_temp_out : ToWorkspace  VariableName=se_hold_inlet_fluid_temp_out  SaveFormat=Structure With Time  SampleTime=-1
  ToWorkspace_se_hold_outlet_fluid_temp_out : ToWorkspace  VariableName=se_hold_outlet_fluid_temp_out  SaveFormat=Structure With Time  SampleTime=-1
  ToWorkspace_shex_buffer_temp_out : ToWorkspace  VariableName=shex_buffer_temp_out  SaveFormat=Structure With Time  SampleTime=-1
  ToWorkspace_sma_hot_buffer_temp_out : ToWorkspace  VariableName=sma_hot_buffer_temp_out  SaveFormat=Structure With Time  SampleTime=-1
  ToWorkspace_sma_stage1_inlet_fluid_temp_out : ToWorkspace  VariableName=sma_stage1_inlet_fluid_temp_out  SaveFormat=Structure With Time  SampleTime=-1
  ToWorkspace_sma_stage1_outlet_fluid_temp_out : ToWorkspace  VariableName=sma_stage1_outlet_fluid_temp_out  SaveFormat=Structure With Time  SampleTime=-1
  ToWorkspace_sma_stage3_inlet_fluid_temp_out : ToWorkspace  VariableName=sma_stage3_inlet_fluid_temp_out  SaveFormat=Structure With Time  SampleTime=-1
  ToWorkspace_sma_stage3_outlet_fluid_temp_out : ToWorkspace  VariableName=sma_stage3_outlet_fluid_temp_out  SaveFormat=Structure With Time  SampleTime=-1
  V1ColdInletColdSideFluidTempPS : nesl_utility/PS-Simulink Converter  PhysicalDomain=network_engine_domain  SubClassName=ps_output  LeftPortType=input  RightPortType=output  PseudoPeriodic=off  Frequencies=[]  VectorFormat=1-D array  Unit=K  AffineConversion=off
      settings: AttributesFormatString=CHEX exchanger retained from mature model
  V1ColdInletColdSideFluidTempSensor : fl_lib/Thermal Liquid/Sensors/Pressure & Temperature Sensor (TL)  reference=foundation.enum.MeasurementReference.absolute  pressure=false  pressure_spec=foundation.enum.PressureMeasementSpec.Absolute  temperature=true
      settings: InternalSimscapePortConfiguration="{\"Bottom\":[{\"id\":\"T\",\"label\":\"T\",\"type\":\"output\"}],\"Left\":[{\"id\":\"A\",\"label\":\"A\",\"type\":\"foundation.thermal_liquid.thermal_liquid\"}],\"Right\":[],\"Top\":[]}"
  V1ColdInletSESideFluidTempPS : nesl_utility/PS-Simulink Converter  PhysicalDomain=network_engine_domain  SubClassName=ps_output  LeftPortType=input  RightPortType=output  PseudoPeriodic=off  Frequencies=[]  VectorFormat=1-D array  Unit=K  AffineConversion=off
      settings: AttributesFormatString=CHEX exchanger retained from mature model
  V1ColdInletSESideFluidTempSensor : fl_lib/Thermal Liquid/Sensors/Pressure & Temperature Sensor (TL)  reference=foundation.enum.MeasurementReference.absolute  pressure=false  pressure_spec=foundation.enum.PressureMeasementSpec.Absolute  temperature=true
      settings: InternalSimscapePortConfiguration="{\"Bottom\":[{\"id\":\"T\",\"label\":\"T\",\"type\":\"output\"}],\"Left\":[{\"id\":\"A\",\"label\":\"A\",\"type\":\"foundation.thermal_liquid.thermal_liquid\"}],\"Right\":[],\"Top\":[]}"
  V1_cold_inlet : SimscapeFluids_lib/Thermal Liquid/Valves & Orifices/Flow Coefficient Parameterized Valve (TL)  flow_coeff_spec=fluids.thermal_liquid.valves.enum.flow_coeff_spec.cv  Cv_max=1  Cv_min=valve_min_Cv  Kv_max=1  Kv_min=valve_min_Cv  valve_character=fluids.thermal_liquid.valves.enum.valve_opening_spec.linear  rangeability=50  alpha=2  area=pipe_fa m^2  Re_c=150  smoothing_factor=0.01
      settings: AttributesFormatString=Retained mature route gate V1  InternalSimscapePortConfiguration="{\"Bottom\":[],\"Left\":[{\"id\":\"A\",\"label\":\"A\",\"type\":\"foundation.thermal_liquid.thermal_liquid\"},{\"id\":\"L\",\"label\":\"L\",\"type\":\"input\"}],\"Right\":[{\"id\":\"B\",\"label\":\"B\",\"type\":\"foundation.thermal_liquid.thermal_liquid\"}],\"Top\":[]}"
  V2_hot_return : SimscapeFluids_lib/Thermal Liquid/Valves & Orifices/Flow Coefficient Parameterized Valve (TL)  flow_coeff_spec=fluids.thermal_liquid.valves.enum.flow_coeff_spec.cv  Cv_max=1  Cv_min=valve_min_Cv  Kv_max=1  Kv_min=valve_min_Cv  valve_character=fluids.thermal_liquid.valves.enum.valve_opening_spec.linear  rangeability=50  alpha=2  area=pipe_fa m^2  Re_c=150  smoothing_factor=0.01
      settings: AttributesFormatString=Retained mature route gate V2  InternalSimscapePortConfiguration="{\"Bottom\":[],\"Left\":[{\"id\":\"A\",\"label\":\"A\",\"type\":\"foundation.thermal_liquid.thermal_liquid\"},{\"id\":\"L\",\"label\":\"L\",\"type\":\"input\"}],\"Right\":[{\"id\":\"B\",\"label\":\"B\",\"type\":\"foundation.thermal_liquid.thermal_liquid\"}],\"Top\":[]}"
  V3SEToHotHotSideFluidTempPS : nesl_utility/PS-Simulink Converter  PhysicalDomain=network_engine_domain  SubClassName=ps_output  LeftPortType=input  RightPortType=output  PseudoPeriodic=off  Frequencies=[]  VectorFormat=1-D array  Unit=K  AffineConversion=off
      settings: AttributesFormatString=HHEX/THE exchanger retained from mature model
  V3SEToHotHotSideFluidTempSensor : fl_lib/Thermal Liquid/Sensors/Pressure & Temperature Sensor (TL)  reference=foundation.enum.MeasurementReference.absolute  pressure=false  pressure_spec=foundation.enum.PressureMeasementSpec.Absolute  temperature=true
      settings: InternalSimscapePortConfiguration="{\"Bottom\":[{\"id\":\"T\",\"label\":\"T\",\"type\":\"output\"}],\"Left\":[{\"id\":\"A\",\"label\":\"A\",\"type\":\"foundation.thermal_liquid.thermal_liquid\"}],\"Right\":[],\"Top\":[]}"
  V3SEToHotSESideFluidTempPS : nesl_utility/PS-Simulink Converter  PhysicalDomain=network_engine_domain  SubClassName=ps_output  LeftPortType=input  RightPortType=output  PseudoPeriodic=off  Frequencies=[]  VectorFormat=1-D array  Unit=K  AffineConversion=off
      settings: AttributesFormatString=HHEX/THE exchanger retained from mature model
  V3SEToHotSESideFluidTempSensor : fl_lib/Thermal Liquid/Sensors/Pressure & Temperature Sensor (TL)  reference=foundation.enum.MeasurementReference.absolute  pressure=false  pressure_spec=foundation.enum.PressureMeasementSpec.Absolute  temperature=true
      settings: InternalSimscapePortConfiguration="{\"Bottom\":[{\"id\":\"T\",\"label\":\"T\",\"type\":\"output\"}],\"Left\":[{\"id\":\"A\",\"label\":\"A\",\"type\":\"foundation.thermal_liquid.thermal_liquid\"}],\"Right\":[],\"Top\":[]}"
  V3_sma_to_hot : SimscapeFluids_lib/Thermal Liquid/Valves & Orifices/Flow Coefficient Parameterized Valve (TL)  flow_coeff_spec=fluids.thermal_liquid.valves.enum.flow_coeff_spec.cv  Cv_max=1  Cv_min=valve_min_Cv  Kv_max=1  Kv_min=valve_min_Cv  valve_character=fluids.thermal_liquid.valves.enum.valve_opening_spec.linear  rangeability=50  alpha=2  area=pipe_fa m^2  Re_c=150  smoothing_factor=0.01
      settings: AttributesFormatString=Retained mature route gate V3  InternalSimscapePortConfiguration="{\"Bottom\":[],\"Left\":[{\"id\":\"A\",\"label\":\"A\",\"type\":\"foundation.thermal_liquid.thermal_liquid\"},{\"id\":\"L\",\"label\":\"L\",\"type\":\"input\"}],\"Right\":[{\"id\":\"B\",\"label\":\"B\",\"type\":\"foundation.thermal_liquid.thermal_liquid\"}],\"Top\":[]}"
  V4HotInletHotSideFluidTempPS : nesl_utility/PS-Simulink Converter  PhysicalDomain=network_engine_domain  SubClassName=ps_output  LeftPortType=input  RightPortType=output  PseudoPeriodic=off  Frequencies=[]  VectorFormat=1-D array  Unit=K  AffineConversion=off
      settings: AttributesFormatString=HHEX/THE exchanger retained from mature model
  V4HotInletHotSideFluidTempSensor : fl_lib/Thermal Liquid/Sensors/Pressure & Temperature Sensor (TL)  reference=foundation.enum.MeasurementReference.absolute  pressure=false  pressure_spec=foundation.enum.PressureMeasementSpec.Absolute  temperature=true
      settings: InternalSimscapePortConfiguration="{\"Bottom\":[{\"id\":\"T\",\"label\":\"T\",\"type\":\"output\"}],\"Left\":[{\"id\":\"A\",\"label\":\"A\",\"type\":\"foundation.thermal_liquid.thermal_liquid\"}],\"Right\":[],\"Top\":[]}"
  V4HotInletSESideFluidTempPS : nesl_utility/PS-Simulink Converter  PhysicalDomain=network_engine_domain  SubClassName=ps_output  LeftPortType=input  RightPortType=output  PseudoPeriodic=off  Frequencies=[]  VectorFormat=1-D array  Unit=K  AffineConversion=off
      settings: AttributesFormatString=HHEX/THE exchanger retained from mature model
  V4HotInletSESideFluidTempSensor : fl_lib/Thermal Liquid/Sensors/Pressure & Temperature Sensor (TL)  reference=foundation.enum.MeasurementReference.absolute  pressure=false  pressure_spec=foundation.enum.PressureMeasementSpec.Absolute  temperature=true
      settings: InternalSimscapePortConfiguration="{\"Bottom\":[{\"id\":\"T\",\"label\":\"T\",\"type\":\"output\"}],\"Left\":[{\"id\":\"A\",\"label\":\"A\",\"type\":\"foundation.thermal_liquid.thermal_liquid\"}],\"Right\":[],\"Top\":[]}"
  V4_hot_inlet : SimscapeFluids_lib/Thermal Liquid/Valves & Orifices/Flow Coefficient Parameterized Valve (TL)  flow_coeff_spec=fluids.thermal_liquid.valves.enum.flow_coeff_spec.cv  Cv_max=1  Cv_min=valve_min_Cv  Kv_max=1  Kv_min=valve_min_Cv  valve_character=fluids.thermal_liquid.valves.enum.valve_opening_spec.linear  rangeability=50  alpha=2  area=pipe_fa m^2  Re_c=150  smoothing_factor=0.01
      settings: AttributesFormatString=Retained mature route gate V4  InternalSimscapePortConfiguration="{\"Bottom\":[],\"Left\":[{\"id\":\"A\",\"label\":\"A\",\"type\":\"foundation.thermal_liquid.thermal_liquid\"},{\"id\":\"L\",\"label\":\"L\",\"type\":\"input\"}],\"Right\":[{\"id\":\"B\",\"label\":\"B\",\"type\":\"foundation.thermal_liquid.thermal_liquid\"}],\"Top\":[]}"
  V5_cold_return : SimscapeFluids_lib/Thermal Liquid/Valves & Orifices/Flow Coefficient Parameterized Valve (TL)  flow_coeff_spec=fluids.thermal_liquid.valves.enum.flow_coeff_spec.cv  Cv_max=1  Cv_min=valve_min_Cv  Kv_max=1  Kv_min=valve_min_Cv  valve_character=fluids.thermal_liquid.valves.enum.valve_opening_spec.linear  rangeability=50  alpha=2  area=pipe_fa m^2  Re_c=150  smoothing_factor=0.01
      settings: AttributesFormatString=Retained mature route gate V5  InternalSimscapePortConfiguration="{\"Bottom\":[],\"Left\":[{\"id\":\"A\",\"label\":\"A\",\"type\":\"foundation.thermal_liquid.thermal_liquid\"},{\"id\":\"L\",\"label\":\"L\",\"type\":\"input\"}],\"Right\":[{\"id\":\"B\",\"label\":\"B\",\"type\":\"foundation.thermal_liquid.thermal_liquid\"}],\"Top\":[]}"
  V6SEToChipChipSideFluidTempPS : nesl_utility/PS-Simulink Converter  PhysicalDomain=network_engine_domain  SubClassName=ps_output  LeftPortType=input  RightPortType=output  PseudoPeriodic=off  Frequencies=[]  VectorFormat=1-D array  Unit=K  AffineConversion=off
  V6SEToChipChipSideFluidTempSensor : fl_lib/Thermal Liquid/Sensors/Pressure & Temperature Sensor (TL)  reference=foundation.enum.MeasurementReference.absolute  pressure=false  pressure_spec=foundation.enum.PressureMeasementSpec.Absolute  temperature=true
      settings: InternalSimscapePortConfiguration="{\"Bottom\":[{\"id\":\"T\",\"label\":\"T\",\"type\":\"output\"}],\"Left\":[{\"id\":\"A\",\"label\":\"A\",\"type\":\"foundation.thermal_liquid.thermal_liquid\"}],\"Right\":[],\"Top\":[]}"
  V6SEToChipSESideFluidTempPS : nesl_utility/PS-Simulink Converter  PhysicalDomain=network_engine_domain  SubClassName=ps_output  LeftPortType=input  RightPortType=output  PseudoPeriodic=off  Frequencies=[]  VectorFormat=1-D array  Unit=K  AffineConversion=off
  V6SEToChipSESideFluidTempSensor : fl_lib/Thermal Liquid/Sensors/Pressure & Temperature Sensor (TL)  reference=foundation.enum.MeasurementReference.absolute  pressure=false  pressure_spec=foundation.enum.PressureMeasementSpec.Absolute  temperature=true
      settings: InternalSimscapePortConfiguration="{\"Bottom\":[{\"id\":\"T\",\"label\":\"T\",\"type\":\"output\"}],\"Left\":[{\"id\":\"A\",\"label\":\"A\",\"type\":\"foundation.thermal_liquid.thermal_liquid\"}],\"Right\":[],\"Top\":[]}"
  V6_sma_to_chip_cold : SimscapeFluids_lib/Thermal Liquid/Valves & Orifices/Flow Coefficient Parameterized Valve (TL)  flow_coeff_spec=fluids.thermal_liquid.valves.enum.flow_coeff_spec.cv  Cv_max=1  Cv_min=valve_min_Cv  Kv_max=1  Kv_min=valve_min_Cv  valve_character=fluids.thermal_liquid.valves.enum.valve_opening_spec.linear  rangeability=50  alpha=2  area=pipe_fa m^2  Re_c=150  smoothing_factor=0.01
      settings: AttributesFormatString=Retained mature route gate V6  InternalSimscapePortConfiguration="{\"Bottom\":[],\"Left\":[{\"id\":\"A\",\"label\":\"A\",\"type\":\"foundation.thermal_liquid.thermal_liquid\"},{\"id\":\"L\",\"label\":\"L\",\"type\":\"input\"}],\"Right\":[{\"id\":\"B\",\"label\":\"B\",\"type\":\"foundation.thermal_liquid.thermal_liquid\"}],\"Top\":[]}"
  ValveCommandFromWorkspace : FromWorkspace  VariableName=L_valve_command  OutputAfterFinalValue=Holding final value
      settings: AttributesFormatString=Four-stage valve command input for route gates
  冷端换热器 : Subsystem
      settings: AttributesFormatString=CHEX exchanger retained from mature model
  热流体设置 : fl_lib/Thermal Liquid/Utilities/Thermal Liquid Settings (TL)  table_dimensions=1  T_TLU=[255.05;283.15;313.15;338.15;363.15;393.15] K  p_TLU=[0.01, 0.1, 5 : 5 : 50] MPa  p_atm=0.5 MPa  pT_region_flag=0  T_min=273.16 K  T_max=405 K  p_min=0.01 MPa  p_max=50 MPa  T_min_1D=255.05 K  T_max_1D=393.15 K  p_min_1D=0.45 MPa  p_max_1D=5 MPa  pT_validity_TLU=[1, 1, 1, 1, 1, 1, 1, 1, 1, 1, 1, 1; 1, 1, 1, 1, 1, 1, 1, 1, 1, 1, 1, 1; 1, 1, 1, 1, 1, 1, 1, 1, 1, 1, 1, 1; 1, 1, 1, 1, 1, 1, 1, 1, 1, 1, 1, 1; 1, 1, 1, 1, 1, 1, 1, 1, 1, 1, 1, 1; 0, 1, 1, 1, 1, 1, 1, 1, 1, 1, 1, 1; 0, 1, 1, 1, 1, 1, 1, 1, 1, 1, 1, 1; 0, 1, 1, 1, 1, 1, 1, 1, 1, 1, 1, 1; 0, 1, 1, 1, 1, 1, 1, 1, 1, 1, 1, 1; 0, 1, 1, 1, 1, 1, 1, 1, 1, 1, 1, 1; 0, 0, 1, 1, 1, 1, 1, 1, 1, 1, 1, 1]  properties_range_check=simscape.enum.assert.action.error  rho_parameterization_2D=1  rho_parameterization_1D=1  rho_TLU=[999.7973, 999.8431, 1002.3216, 1004.8218, 1007.293, 1009.7358, 1012.1506, 1014.5379, 1016.8979, 1019.2311, 1021.538, 1023.8188; 999.6579, 999.7009, 1002.0303, 1004.382, 1006.7084, 1009.0101, 1011.2874, 1013.5407, 1015.7703, 1017.9766, 1020.1599, 1022.3206; 998.1632, 998.2045, 1000.4375, 1002.6924, 1004.9239, 1007.1324, 1009.3183, 1011.4819, 1013.6236, 1015.7438, 1017.8428, 1019.921; 995.6057, 995.6458, 997.81864, 1000.0128, 1002.1841, 1004.3332, 1006.4603, 1008.566, 1010.6505, 1012.7144, 1014.758, 1016.7815; 992.1724, 992.2119, 994.35133, 996.5113, 998.6484, 1000.7633, 1002.8563, 1004.928, 1006.9788, 1009.009, 1011.0192, 1013.0097; 988.02, 988.0299, 990.15684, 992.3035, 994.4268, 996.5273, 998.6056, 1000.6622, 1002.6976, 1004.7123, 1006.7067, 1008.6813; 983.18, 983.1901, 985.3217, 987.4721, 989.5983, 991.7008, 993.7803, 995.8374, 997.8726, 999.8864, 1001.8795, 1003.8522; 977.75, 977.7583, 979.9094, 982.0783, 984.2216, 986.34, 988.4343, 990.505, 992.5529, 994.5786, 996.5825, 998.5654; 971.77, 971.7836, 973.96734, 976.1678, 978.3409, 980.4876, 982.6087, 984.7049, 986.7768, 988.8254, 990.8511, 992.8545; 965.26, 965.3023, 967.53107, 969.7753, 971.9901, 974.1764, 976.3354, 978.4676, 980.5741, 982.6556, 984.7129, 986.7465; 958.62, 958.6315, 960.627, 962.9267, 965.1944, 967.4314, 969.6387, 971.8173, 973.9681, 976.0921, 978.19, 980.2628] kg/m^3  beta_TLU=[1.9649, 1.9654, 1.9929, 2.0213, 2.0499, 2.0787, 2.1078, 2.1372, 2.1668, 2.1966, 2.2268, 2.2572; 2.0913, 2.0918, 2.1191, 2.1471, 2.1752, 2.2036, 2.2322, 2.261, 2.2899, 2.3191, 2.3485, 2.3781; 2.1786, 2.1791, 2.2067, 2.235, 2.2634, 2.2919, 2.3206, 2.3494, 2.3784, 2.4075, 2.4367, 2.4661; 2.2332, 2.2337, 2.2619, 2.2908, 2.3197, 2.3487, 2.3778, 2.407, 2.4363, 2.4657, 2.4951, 2.5246; 2.26, 2.2605, 2.2895, 2.3191, 2.3487, 2.3784, 2.4081, 2.4378, 2.4675, 2.4973, 2.5272, 2.5571; 2.2638, 2.2638, 2.2936, 2.324, 2.3544, 2.3848, 2.4151, 2.4455, 2.4758, 2.5062, 2.5365, 2.5669; 2.2472, 2.2472, 2.2779, 2.3092, 2.3403, 2.3715, 2.4025, 2.4336, 2.4646, 2.4955, 2.5264, 2.5573; 2.214, 2.214, 2.2455, 2.2776, 2.3096, 2.3415, 2.3733, 2.405, 2.4367, 2.4683, 2.4998, 2.5313; 2.1668, 2.1668, 2.1992, 2.2321, 2.2649, 2.2976, 2.3301, 2.3626, 2.3949, 2.4272, 2.4593, 2.4914; 2.1081, 2.1081, 2.1413, 2.175, 2.2086, 2.2421, 2.2754, 2.3085, 2.3415, 2.3744, 2.4072, 2.4399; 2.0494, 2.0494, 2.0739, 2.1084, 2.1428, 2.177, 2.211, 2.2449, 2.2786, 2.3121, 2.3455, 2.3788] GPa  alpha_TLU=1e-4 * [-.679, -.676, -.49, -.307, -.13, .041, .206, .365, .519, .668, .811, .949; .878, .881, .998, 1.114, 1.227, 1.337, 1.445, 1.549, 1.651, 1.75, 1.846, 1.939; 2.068, 2.069, 2.141, 2.213, 2.283, 2.352, 2.42, 2.486, 2.551, 2.614, 2.676, 2.736; 3.034, 3.035, 3.074, 3.113, 3.152, 3.191, 3.229, 3.267, 3.305, 3.341, 3.377, 3.413; 3.855, 3.856, 3.87, 3.884, 3.899, 3.914, 3.93, 3.946, 3.961, 3.977, 3.993, 4.009; 4.578, 4.578, 4.572, 4.566, 4.562, 4.558, 4.555, 4.552, 4.55, 4.549, 4.548, 4.547; 5.233, 5.233, 5.209, 5.186, 5.165, 5.144, 5.125, 5.107, 5.09, 5.074, 5.059, 5.045; 5.84, 5.84, 5.801, 5.762, 5.725, 5.691, 5.657, 5.625, 5.595, 5.566, 5.538, 5.512; 6.414, 6.414, 6.36, 6.307, 6.256, 6.208, 6.161, 6.117, 6.074, 6.033, 5.994, 5.956; 6.967, 6.967, 6.898, 6.831, 6.766, 6.705, 6.646, 6.589, 6.535, 6.482, 6.432, 6.384; 7.519, 7.519, 7.423, 7.342, 7.264, 7.189, 7.118, 7.049, 6.983, 6.92, 6.859, 6.8] 1/K  rho_TLU_2=[999.7973, 999.8431, 1002.3216, 1004.8218, 1007.293, 1009.7358, 1012.1506, 1014.5379, 1016.8979, 1019.2311, 1021.538, 1023.8188; 999.6579, 999.7009, 1002.0303, 1004.382, 1006.7084, 1009.0101, 1011.2874, 1013.5407, 1015.7703, 1017.9766, 1020.1599, 1022.3206; 998.1632, 998.2045, 1000.4375, 1002.6924, 1004.9239, 1007.1324, 1009.3183, 1011.4819, 1013.6236, 1015.7438, 1017.8428, 1019.921; 995.6057, 995.6458, 997.81864, 1000.0128, 1002.1841, 1004.3332, 1006.4603, 1008.566, 1010.6505, 1012.7144, 1014.758, 1016.7815; 992.1724, 992.2119, 994.35133, 996.5113, 998.6484, 1000.7633, 1002.8563, 1004.928, 1006.9788, 1009.009, 1011.0192, 1013.0097; 988.02, 988.0299, 990.15684, 992.3035, 994.4268, 996.5273, 998.6056, 1000.6622, 1002.6976, 1004.7123, 1006.7067, 1008.6813; 983.18, 983.1901, 985.3217, 987.4721, 989.5983, 991.7008, 993.7803, 995.8374, 997.8726, 999.8864, 1001.8795, 1003.8522; 977.75, 977.7583, 979.9094, 982.0783, 984.2216, 986.34, 988.4343, 990.505, 992.5529, 994.5786, 996.5825, 998.5654; 971.77, 971.7836, 973.96734, 976.1678, 978.3409, 980.4876, 982.6087, 984.7049, 986.7768, 988.8254, 990.8511, 992.8545; 965.26, 965.3023, 967.53107, 969.7753, 971.9901, 974.1764, 976.3354, 978.4676, 980.5741, 982.6556, 984.7129, 986.7465; 958.62, 958.6315, 960.627, 962.9267, 965.1944, 967.4314, 969.6387, 971.8173, 973.9681, 976.0921, 978.19, 980.2628] kg/m^3  rho_ref_3=998.21 kg/m^3  T_ref_3=293.16 K  p_ref_3=0.101325 MPa  beta_const_3=2.1791 GPa  alpha_const_3=2.0691e-4 1/K  rho_TLU_4=[1066.03926666667;1055.38;1039.77;1023.55;1004.39;977.53] kg/m^3  beta_const_4=2 GPa  p_ref_4=0.5 MPa  rho_ref_5=998.21 kg/m^3  T_ref_5=293.16 K  p_ref_5=0.101325 MPa  beta_const_5=2.1791 GPa  alpha_const_5=2.0691e-4 1/K  u_parameterization_2D=1  u_parameterization_1D=1  u_TLU=[.0002, .0018, .086, .1588, .219, .267, .3034, .3288, .3436, .3483, .3435, .3294; 42.062, 42.06, 41.935, 41.804, 41.668, 41.527, 41.382, 41.233, 41.081, 40.924, 40.763, 40.599; 83.953, 83.948, 83.651, 83.349, 83.049, 82.749, 82.451, 82.153, 81.856, 81.56, 81.265, 80.971; 125.77, 125.76, 125.31, 124.86, 124.41, 123.97, 123.53, 123.1, 122.68, 122.25, 121.84, 121.42; 167.57, 167.56, 166.96, 166.37, 165.79, 165.21, 164.65, 164.09, 163.54, 163, 162.46, 161.94; 209.36, 209.36, 208.63, 207.9, 207.19, 206.48, 205.79, 205.11, 204.45, 203.79, 203.14, 202.5; 251.19, 251.19, 250.33, 249.47, 248.62, 247.79, 246.98, 246.18, 245.39, 244.62, 243.86, 243.12; 293.06, 293.06, 292.07, 291.07, 290.1, 289.14, 288.2, 287.28, 286.38, 285.49, 284.62, 283.77; 334.99, 334.99, 333.86, 332.73, 331.63, 330.54, 329.48, 328.44, 327.41, 326.41, 325.43, 324.46; 377, 377, 375.73, 374.46, 373.22, 372, 370.81, 369.64, 368.5, 367.38, 366.27, 365.19; 419.01, 419.01, 417.69, 416.27, 414.89, 413.54, 412.21, 410.91, 409.64, 408.4, 407.17, 405.98] kJ/kg  cp_TLU=[4.2199, 4.2194, 4.1957, 4.1726, 4.1508, 4.13, 4.1103, 4.0916, 4.0738, 4.0569, 4.0408, 4.0254; 4.1955, 4.1951, 4.1769, 4.1592, 4.1422, 4.1259, 4.1103, 4.0954, 4.0812, 4.0676, 4.0545, 4.0421; 4.1843, 4.184, 4.169, 4.1543, 4.1401, 4.1264, 4.1133, 4.1007, 4.0885, 4.0768, 4.0656, 4.0548; 4.1801, 4.1798, 4.1667, 4.1538, 4.1413, 4.1293, 4.1177, 4.1064, 4.0956, 4.0851, 4.075, 4.0653; 4.1796, 4.1794, 4.1675, 4.1558, 4.1444, 4.1334, 4.1227, 4.1123, 4.1023, 4.0926, 4.0832, 4.0741; 4.1813, 4.1813, 4.1702, 4.1592, 4.1484, 4.138, 4.1279, 4.1181, 4.1086, 4.0993, 4.0903, 4.0816; 4.185, 4.185, 4.1742, 4.1636, 4.1532, 4.1432, 4.1334, 4.1239, 4.1146, 4.1056, 4.0969, 4.0884; 4.1901, 4.1901, 4.1795, 4.169, 4.1588, 4.1489, 4.1393, 4.1299, 4.1207, 4.1118, 4.1032, 4.0947; 4.1968, 4.1968, 4.1862, 4.1757, 4.1655, 4.1555, 4.1458, 4.1364, 4.1273, 4.1183, 4.1096, 4.1012; 4.2052, 4.2052, 4.1944, 4.1837, 4.1733, 4.1632, 4.1534, 4.1438, 4.1345, 4.1255, 4.1166, 4.108; 4.2136, 4.2136, 4.2045, 4.1935, 4.1828, 4.1724, 4.1623, 4.1524, 4.1429, 4.1335, 4.1245, 4.1157] kJ/kg/K  u_TLU_2=[.0002, .0018, .086, .1588, .219, .267, .3034, .3288, .3436, .3483, .3435, .3294; 42.062, 42.06, 41.935, 41.804, 41.668, 41.527, 41.382, 41.233, 41.081, 40.924, 40.763, 40.599; 83.953, 83.948, 83.651, 83.349, 83.049, 82.749, 82.451, 82.153, 81.856, 81.56, 81.265, 80.971; 125.77, 125.76, 125.31, 124.86, 124.41, 123.97, 123.53, 123.1, 122.68, 122.25, 121.84, 121.42; 167.57, 167.56, 166.96, 166.37, 165.79, 165.21, 164.65, 164.09, 163.54, 163, 162.46, 161.94; 209.36, 209.36, 208.63, 207.9, 207.19, 206.48, 205.79, 205.11, 204.45, 203.79, 203.14, 202.5; 251.19, 251.19, 250.33, 249.47, 248.62, 247.79, 246.98, 246.18, 245.39, 244.62, 243.86, 243.12; 293.06, 293.06, 292.07, 291.07, 290.1, 289.14, 288.2, 287.28, 286.38, 285.49, 284.62, 283.77; 334.99, 334.99, 333.86, 332.73, 331.63, 330.54, 329.48, 328.44, 327.41, 326.41, 325.43, 324.46; 377, 377, 375.73, 374.46, 373.22, 372, 370.81, 369.64, 368.5, 367.38, 366.27, 365.19; 419.01, 419.01, 417.69, 416.27, 414.89, 413.54, 412.21, 410.91, 409.64, 408.4, 407.17, 405.98] kJ/kg  cp_TLU_3=[4.2199, 4.2194, 4.1957, 4.1726, 4.1508, 4.13, 4.1103, 4.0916, 4.0738, 4.0569, 4.0408, 4.0254; 4.1955, 4.1951, 4.1769, 4.1592, 4.1422, 4.1259, 4.1103, 4.0954, 4.0812, 4.0676, 4.0545, 4.0421; 4.1843, 4.184, 4.169, 4.1543, 4.1401, 4.1264, 4.1133, 4.1007, 4.0885, 4.0768, 4.0656, 4.0548; 4.1801, 4.1798, 4.1667, 4.1538, 4.1413, 4.1293, 4.1177, 4.1064, 4.0956, 4.0851, 4.075, 4.0653; 4.1796, 4.1794, 4.1675, 4.1558, 4.1444, 4.1334, 4.1227, 4.1123, 4.1023, 4.0926, 4.0832, 4.0741; 4.1813, 4.1813, 4.1702, 4.1592, 4.1484, 4.138, 4.1279, 4.1181, 4.1086, 4.0993, 4.0903, 4.0816; 4.185, 4.185, 4.1742, 4.1636, 4.1532, 4.1432, 4.1334, 4.1239, 4.1146, 4.1056, 4.0969, 4.0884; 4.1901, 4.1901, 4.1795, 4.169, 4.1588, 4.1489, 4.1393, 4.1299, 4.1207, 4.1118, 4.1032, 4.0947; 4.1968, 4.1968, 4.1862, 4.1757, 4.1655, 4.1555, 4.1458, 4.1364, 4.1273, 4.1183, 4.1096, 4.1012; 4.2052, 4.2052, 4.1944, 4.1837, 4.1733, 4.1632, 4.1534, 4.1438, 4.1345, 4.1255, 4.1166, 4.108; 4.2136, 4.2136, 4.2045, 4.1935, 4.1828, 4.1724, 4.1623, 4.1524, 4.1429, 4.1335, 4.1245, 4.1157] kJ/kg/K  u_TLU_4=[0;98.6876214999999;207.2726215;300.2976215;395.6226215;513.0576215] kJ/kg  cp_TLU_5=[4.2199; 4.1955; 4.1843; 4.1801; 4.1796; 4.1813; 4.185; 4.1901; 4.1968; 4.2052; 4.2136] kJ/kg/K  nu_TLU=[1.7917, 1.7914, 1.7763, 1.7615, 1.7473, 1.7338, 1.7208, 1.7085, 1.6967, 1.6854, 1.6747, 1.6645; 1.3061, 1.3059, 1.2986, 1.2914, 1.2845, 1.2779, 1.2716, 1.2656, 1.2598, 1.2543, 1.2491, 1.2441; 1.0032, 1.0032, .9995, .9959, .9924, .9891, .9859, .9829, .9801, .9774, .9748, .9724; .8006, .8005, .7987, .797, .7953, .7937, .7922, .7908, .7894, .7881, .787, .7859; .6577, .6577, .657, .6562, .6555, .6548, .6543, .6537, .6532, .6528, .6523, .652; .553, .553, .5529, .5527, .5526, .5525, .5524, .5524, .5524, .5524, .5524, .5525; .4739, .4739, .4741, .4743, .4745, .4747, .475, .4753, .4755, .4758, .4762, .4765; .4127, .4127, .4131, .4135, .4139, .4143, .4148, .4152, .4157, .4162, .4167, .4172; .3643, .3643, .3648, .3654, .3659, .3665, .367, .3676, .3682, .3688, .3694, .37; .3254, .3254, .3261, .3267, .3273, .328, .3286, .3293, .3299, .3306, .3312, .3319; .2866, .2866, .2945, .2952, .2959, .2965, .2972, .2979, .2986, .2993, .3, .3007] mm^2/s  nu_TLU_2=[40.6392421106322;6.83857946900642;2.15326466430076;1.14913780469933;0.742938499985066;0.520086340061174] mm^2/s  k_TLU=[561.04, 561.09, 563.8, 566.56, 569.32, 572.08, 574.82, 577.54, 580.24, 582.92, 585.57, 588.18; 580.02, 580.07, 582.45, 584.88, 587.32, 589.75, 592.18, 594.61, 597.02, 599.42, 601.8, 604.16; 598.44, 598.48, 600.73, 603.03, 605.33, 607.64, 609.94, 612.24, 614.54, 616.82, 619.1, 621.36; 615.48, 615.52, 617.73, 620, 622.26, 624.54, 626.81, 629.07, 631.34, 633.6, 635.85, 638.09; 630.6, 630.64, 632.87, 635.15, 637.44, 639.72, 642.01, 644.29, 646.57, 648.84, 651.11, 653.36; 643.61, 643.61, 645.88, 648.21, 650.53, 652.86, 655.18, 657.51, 659.82, 662.14, 664.44, 666.74; 654.39, 654.39, 656.73, 659.12, 661.5, 663.89, 666.27, 668.65, 671.02, 673.38, 675.74, 678.09; 663.13, 663.13, 665.54, 668, 670.46, 672.91, 675.36, 677.8, 680.24, 682.67, 685.09, 687.5; 670.02, 670.02, 672.51, 675.05, 677.59, 680.12, 682.64, 685.16, 687.67, 690.17, 692.66, 695.14; 675.27, 675.27, 677.85, 680.48, 683.11, 685.73, 688.34, 690.94, 693.53, 696.11, 698.68, 701.24; 680.52, 680.52, 681.77, 684.5, 687.22, 689.94, 692.64, 695.34, 698.02, 700.69, 703.35, 706] mW/m/K  k_TLU_2=[365.406333333333;393.6;415;426.2;431.3;429.4] mW/m/K
  热端换热器 : Subsystem
      settings: AttributesFormatString=HHEX/THE exchanger retained from mature model
  wires:
  PS-Simulink Converter2/1 -> Scope/1
  PS-Simulink Converter3/1 -> Scope1/1
  Demux/1 -> MATLAB Function/1(v1_cold_inlet), Simulink-PS Converter/1
  Demux/2 -> MATLAB Function/2(v2_hot_return), Simulink-PS Converter1/1
  Demux/3 -> MATLAB Function/4(v4_hot_inlet), Simulink-PS Converter2/1
  Demux/4 -> MATLAB Function/3(v3_sma_to_hot), Simulink-PS Converter3/1
  Demux/5 -> MATLAB Function/5(v5_cold_return), Simulink-PS Converter4/1
  Demux/6 -> MATLAB Function/6(v6_sma_to_chip_cold), Simulink-PS Converter5/1
  MATLAB Function/1(y) -> ?
  ValveCommandFromWorkspace/1 -> Demux/1
  FlowSensor_V1_cold_inlet_PS/1 -> ToWorkspace_mass_flow_v1_cold_inlet_kgps/1, PressurePI_PassthruV1/1
  FlowSensor_V3_sma_to_hot_PS/1 -> ToWorkspace_mass_flow_v3_sma_to_hot_kgps/1
  FlowSensor_V4_hot_inlet_PS/1 -> ToWorkspace_mass_flow_v4_hot_inlet_kgps/1, PressurePI_PassthruV4/1
  FlowSensor_V6_sma_to_chip_cold_PS/1 -> ToWorkspace_mass_flow_v6_sma_to_chip_cold_kgps/1
  HotFluidBufferTempPS/1 -> ToWorkspace_hot_buffer_temp_out/1, ToWorkspace_probe_root_hot_buffer_fluid_T_K/1
  ColdFluidBufferTempPS/1 -> ToWorkspace_cold_buffer_temp_out/1, ToWorkspace_probe_root_cold_buffer_fluid_T_K/1
  SEHoldInletFluidTempPS/1 -> ToWorkspace_se_hold_inlet_fluid_temp_out/1, ToWorkspace_probe_sma_stage2_port1_v1_side_T_K/1
  SEHoldOutletFluidTempPS/1 -> ToWorkspace_se_hold_outlet_fluid_temp_out/1, ToWorkspace_probe_sma_stage2_port2_v3_side_T_K/1
  SECooldownInletFluidTempPS/1 -> ToWorkspace_se_cooldown_inlet_fluid_temp_out/1, ToWorkspace_probe_sma_stage4_port3_v4_side_T_K/1
  SECooldownOutletFluidTempPS/1 -> ToWorkspace_se_cooldown_outlet_fluid_temp_out/1, ToWorkspace_probe_sma_stage4_port4_v6_side_T_K/1
  V1ColdInletColdSideFluidTempPS/1 -> ToWorkspace_probe_v1_cold_inlet_cold_buffer_side_T_K/1
  V1ColdInletSESideFluidTempPS/1 -> ToWorkspace_probe_v1_cold_inlet_sma_side_T_K/1
  V3SEToHotSESideFluidTempPS/1 -> ToWorkspace_probe_v3_sma_to_hot_sma_side_T_K/1
  V3SEToHotHotSideFluidTempPS/1 -> ToWorkspace_probe_v3_sma_to_hot_hot_hx_side_T_K/1
  V4HotInletHotSideFluidTempPS/1 -> ToWorkspace_probe_v4_hot_inlet_hot_buffer_side_T_K/1
  V4HotInletSESideFluidTempPS/1 -> ToWorkspace_probe_v4_hot_inlet_sma_side_T_K/1
  V6SEToChipSESideFluidTempPS/1 -> ToWorkspace_probe_v6_sma_to_chip_sma_side_T_K/1
  V6SEToChipChipSideFluidTempPS/1 -> ToWorkspace_probe_v6_sma_to_chip_chip_side_T_K/1
  PressurePI_TargetCooldown/1 -> PressurePI_ErrorSum/2
  PressurePI_PassthruV1/1 -> PressurePI_ErrorSum/3
  PressurePI_PassthruV4/1 -> PressurePI_ErrorSum/4
  PressurePI_ErrorSum/1 -> PressurePI_ErrorNormalizer/1
  PressurePI_ErrorNormalizer/1 -> PressurePI_ErrorLag/1
  PressurePI_ErrorLag/1 -> PressurePI_Kp/1, PressurePI_Ki/1
  PressurePI_BiasSum/1 -> PressurePI_Saturation/1
  PressurePI_Saturation/1 -> PressurePI_SimulinkPS/1, ToWorkspace_pressure_command_se_MPa/1
  SMAValveCommandFromWorkspace/1 -> SMA_Demux/1
  SMA_Demux/1 -> SMAValveCmdPS1/1
  SMA_Demux/2 -> SMAValveCmdPS2/1
  SMA_Demux/3 -> SMAValveCmdPS3/1
  SMA_Demux/4 -> SMAValveCmdPS4/1
  SMA_Demux/5 -> SMAValveCmdPS5/1
  SMA_Demux/6 -> SMAValveCmdPS6/1
  SMAPressurePI_TargetStage1/1 -> SMAPressurePI_TargetSum/1
  SMAPressurePI_TargetStage3/1 -> SMAPressurePI_TargetSum/2
  FlowSensor_SMA_stage13_loop_PS/1 -> SMAPressurePI_ErrorSum/2, ToWorkspace_mass_flow_sma_stage13_kgps/1
  SMAPressurePI_ErrorSum/1 -> SMAPressurePI_ErrorNormalizer/1
  SMAPressurePI_ErrorNormalizer/1 -> SMAPressurePI_ErrorLag/1
  SMAPressurePI_ErrorLag/1 -> SMAPressurePI_Kp/1, SMAPressurePI_Ki/1
  SMAPressurePI_Ki/1 -> SMAPressurePI_Integrator/1
  SMAPressurePI_Integrator/1 -> SMAPressurePI_BiasSum/2
  SMAPressurePI_BiasSum/1 -> SMAPressurePI_Saturation/1
  SMAPressurePI_Saturation/1 -> SMAPressurePI_SimulinkPS/1, ToWorkspace_pressure_command_sma_MPa/1
  ECC_Constitutive21_Clock/1 -> ECC_Constitutive21_InputMux/1
  ECC_Constitutive21_StateDelay/1 -> ECC_Constitutive21_InputMux/4
  ECC_Constitutive21_InputMux/1 -> ECC_Constitutive21_VectorStep/1
  ECC_Constitutive21_VectorStep/1 -> ECC_Constitutive21_OutputDemux/1, ToWorkspace_ECC_Constitutive21_Output/1
  ECC_Constitutive21_OutputDemux/1 -> ToWorkspace_ECC_Q_SMA_constitutive_W/1, SMA/1(ConstitutiveHeat21_W)
  ECC_Constitutive21_OutputDemux/2 -> ToWorkspace_ECC_Q_SE_constitutive_W/1, SE/1(ConstitutiveHeat21_W)
  ECC_Constitutive21_OutputDemux/3 -> ECC_Constitutive21_StateDelay/1
  ? -> ?
  ? -> ?
  SMAHotFluidBufferTempPS/1 -> ToWorkspace_sma_hot_buffer_temp_out/1
  PressurePI_Kp/1 -> SEPressurePEnableProduct/1
  SEPressureFeedbackEnableFromWorkspace/1 -> SEPressurePEnableProduct/2
  SMAPressurePI_Kp/1 -> SMAPressurePEnableProduct/1
  SMAPressureFeedbackEnableFromWorkspace/1 -> SMAPressurePEnableProduct/2
  FlowSensor_SMA_stage1_route_PS/1 -> ToWorkspace_mass_flow_sma_stage1_route_kgps/1
  FlowSensor_SMA_stage3_route_PS/1 -> ToWorkspace_mass_flow_sma_stage3_route_kgps/1
  SMAPressureBiasFromWorkspace/1 -> SMAPressurePI_BiasSum/3
  SMAFlowTargetFromWorkspace/1 -> SMAPressurePI_ErrorSum/1
  SMAPressurePEnableProduct/1 -> SMAPressurePI_BiasSum/1
  SMAPressureFeedbackResetFromWorkspace/1 -> SMAPressurePI_Integrator/2
  SEPressureBiasFromWorkspace/1 -> PressurePI_BiasSum/3
  SEFlowTargetFromWorkspace/1 -> PressurePI_ErrorSum/1
  SEPressurePEnableProduct/1 -> PressurePI_BiasSum/1
  PressurePI_Ki/1 -> SEStage2PressureIInputGate/1, SEStage4PressureIInputGate/1
  SEStage2PressureIEnableFromWorkspace/1 -> SEStage2PressureIInputGate/2, SEStage2PressureIOutputGate/2
  SEStage2PressureIInputGate/1 -> SEStage2PressurePI_Integrator/1
  SEStage2PressurePI_Integrator/1 -> SEStage2PressureIOutputGate/1
  SEStage4PressureIEnableFromWorkspace/1 -> SEStage4PressureIInputGate/2, SEStage4PressureIOutputGate/2
  SEStage4PressureIInputGate/1 -> SEStage4PressurePI_Integrator/1
  SEStage4PressurePI_Integrator/1 -> SEStage4PressureIOutputGate/1
  SEStage2PressureIOutputGate/1 -> SERoutePressureISum/1
  SEStage4PressureIOutputGate/1 -> SERoutePressureISum/2
  SERoutePressureISum/1 -> PressurePI_BiasSum/2
  SMA/1(NodeTemp21Out) -> ECC_Constitutive21_SMA_TempDelay/1
  ECC_Constitutive21_SMA_TempDelay/1 -> ECC_Constitutive21_InputMux/2
  SE/1(NodeTemp21Out) -> ECC_Constitutive21_SE_TempDelay/1
  ECC_Constitutive21_SE_TempDelay/1 -> ECC_Constitutive21_InputMux/3
  SHEXBufferFluidTempPS/1 -> ToWorkspace_probe_root_shex_buffer_fluid_T_K/1, ToWorkspace_shex_buffer_temp_out/1
  SMAStage1V1SHEXSideFluidTempPS/1 -> ToWorkspace_probe_sma_stage1_v1_shex_side_T_K/1
  SMAStage1V1PumpSideFluidTempPS/1 -> ToWorkspace_probe_sma_stage1_v1_pump_side_T_K/1
  SMAStage13PumpOutletFluidTempPS/1 -> ToWorkspace_probe_sma_stage13_pump_outlet_T_K/1
  SMAStage1InletFluidTempPS/1 -> ToWorkspace_sma_stage1_inlet_fluid_temp_out/1, ToWorkspace_probe_sma_stage1_port1_v3_side_T_K/1
  SMAStage1OutletFluidTempPS/1 -> ToWorkspace_sma_stage1_outlet_fluid_temp_out/1, ToWorkspace_probe_sma_stage1_port2_v5_side_T_K/1
  SMAStage1V5SHEXSideFluidTempPS/1 -> ToWorkspace_probe_sma_stage1_v5_shex_side_T_K/1
  SMAStage3V2HHEXSideFluidTempPS/1 -> ToWorkspace_probe_sma_stage3_v2_hhex_side_T_K/1
  SMAStage3V2PumpSideFluidTempPS/1 -> ToWorkspace_probe_sma_stage3_v2_pump_side_T_K/1
  SMAStage3InletFluidTempPS/1 -> ToWorkspace_sma_stage3_inlet_fluid_temp_out/1, ToWorkspace_probe_sma_stage3_port3_v4_side_T_K/1
  SMAStage3OutletFluidTempPS/1 -> ToWorkspace_sma_stage3_outlet_fluid_temp_out/1, ToWorkspace_probe_sma_stage3_port4_v6_side_T_K/1
  SMAStage3V6HHEXSideFluidTempPS/1 -> ToWorkspace_probe_sma_stage3_v6_hhex_side_T_K/1
  connections:
  Pressure & Temperature Sensor (TL)/RConn1 -- PS-Simulink Converter2/LConn1
  Pressure & Temperature Sensor (TL)1/RConn1 -- PS-Simulink Converter3/LConn1
  ?
  冷端换热器/LConn1 -- V5_cold_return/RConn1
  热端换热器/RConn1 -- V2_hot_return/RConn1
  Simulink-PS Converter/RConn1 -- V1_cold_inlet/LConn2
  Simulink-PS Converter1/RConn1 -- V2_hot_return/LConn2
  Simulink-PS Converter2/RConn1 -- V3_sma_to_hot/LConn2
  Simulink-PS Converter5/RConn1 -- V4_hot_inlet/LConn2
  Simulink-PS Converter4/RConn1 -- V5_cold_return/LConn2
  Simulink-PS Converter3/RConn1 -- V6_sma_to_chip_cold/LConn2
  V3_sma_to_hot/RConn1 -- 热端换热器/LConn1 -- V3SEToHotHotSideFluidTempSensor/LConn1
  冷端换热器/RConn1 -- V6_sma_to_chip_cold/RConn1 -- V6SEToChipChipSideFluidTempSensor/LConn1
  FlowSensor_V1_cold_inlet/LConn1 -- V1_cold_inlet/RConn1 -- V1ColdInletSESideFluidTempSensor/LConn1
  SE/LConn1 -- FlowSensor_V1_cold_inlet/RConn1 -- SEHoldInletFluidTempSensor/LConn1
  FlowSensor_V1_cold_inlet/RConn2 -- FlowSensor_V1_cold_inlet_PS/LConn1
  FlowSensor_V3_sma_to_hot/LConn1 -- SE/LConn2 -- SEHoldOutletFluidTempSensor/LConn1
  V3_sma_to_hot/LConn1 -- FlowSensor_V3_sma_to_hot/RConn1 -- V3SEToHotSESideFluidTempSensor/LConn1
  FlowSensor_V3_sma_to_hot/RConn2 -- FlowSensor_V3_sma_to_hot_PS/LConn1
  FlowSensor_V4_hot_inlet/LConn1 -- V4_hot_inlet/RConn1 -- V4HotInletSESideFluidTempSensor/LConn1
  SE/LConn3 -- FlowSensor_V4_hot_inlet/RConn1 -- SECooldownInletFluidTempSensor/LConn1
  FlowSensor_V4_hot_inlet/RConn2 -- FlowSensor_V4_hot_inlet_PS/LConn1
  FlowSensor_V6_sma_to_chip_cold/LConn1 -- SE/LConn4 -- SECooldownOutletFluidTempSensor/LConn1
  V6_sma_to_chip_cold/LConn1 -- FlowSensor_V6_sma_to_chip_cold/RConn1 -- V6SEToChipSESideFluidTempSensor/LConn1
  FlowSensor_V6_sma_to_chip_cold/RConn2 -- FlowSensor_V6_sma_to_chip_cold_PS/LConn1
  HotFluidBufferTempSensor/RConn1 -- HotFluidBufferTempPS/LConn1
  ColdFluidBufferTempSensor/RConn1 -- ColdFluidBufferTempPS/LConn1
  SEHoldInletFluidTempSensor/RConn1 -- SEHoldInletFluidTempPS/LConn1
  SEHoldOutletFluidTempSensor/RConn1 -- SEHoldOutletFluidTempPS/LConn1
  SECooldownInletFluidTempSensor/RConn1 -- SECooldownInletFluidTempPS/LConn1
  SECooldownOutletFluidTempSensor/RConn1 -- SECooldownOutletFluidTempPS/LConn1
  V1ColdInletColdSideFluidTempSensor/RConn1 -- V1ColdInletColdSideFluidTempPS/LConn1
  V1ColdInletSESideFluidTempSensor/RConn1 -- V1ColdInletSESideFluidTempPS/LConn1
  V3SEToHotSESideFluidTempSensor/RConn1 -- V3SEToHotSESideFluidTempPS/LConn1
  V3SEToHotHotSideFluidTempSensor/RConn1 -- V3SEToHotHotSideFluidTempPS/LConn1
  V4HotInletHotSideFluidTempSensor/RConn1 -- V4HotInletHotSideFluidTempPS/LConn1
  V4HotInletSESideFluidTempSensor/RConn1 -- V4HotInletSESideFluidTempPS/LConn1
  V6SEToChipSESideFluidTempSensor/RConn1 -- V6SEToChipSESideFluidTempPS/LConn1
  V6SEToChipChipSideFluidTempSensor/RConn1 -- V6SEToChipChipSideFluidTempPS/LConn1
  SE_Stage4_PistonPressureSource/LConn2 -- PressurePI_SimulinkPS/RConn1 -- SE_Stage2_PistonPressureSource/LConn2
  SMAValveCmdPS1/RConn1 -- SMA_V1_SHEX_to_pump/LConn2
  SMAValveCmdPS2/RConn1 -- SMA_V2_HHEX_to_pump/LConn2
  SMAValveCmdPS3/RConn1 -- SMA_V3_pump_to_heat_path/LConn2
  SMAValveCmdPS4/RConn1 -- SMA_V4_pump_to_cool_path/LConn2
  SMAValveCmdPS5/RConn1 -- SMA_V5_SMA_to_SHEX/LConn2
  SMAValveCmdPS6/RConn1 -- SMA_V6_SMA_to_HHEX/LConn2
  SMAPressurePI_SimulinkPS/RConn1 -- SMA Pressure Source (TL)/LConn2
  FlowSensor_SMA_stage13_loop/RConn2 -- FlowSensor_SMA_stage13_loop_PS/LConn1
  SHEX/LConn1 -- SHEXFluidBuffer/LConn1 -- SHEXBufferFluidTempSensor/LConn1 -- SMA_V1_SHEX_to_pump/LConn1 -- SMAStage1V1SHEXSideFluidTempSensor/LConn1
  SMA Pressure Source (TL)/RConn1 -- FlowSensor_SMA_stage13_loop/LConn1
  SMA_ThermalLiquidSettings/RConn1 -- 热端换热器/LConn2 -- SMAHotFluidBuffer/LConn1 -- SMAHotFluidBufferTempSensor/LConn1 -- SMA_V2_HHEX_to_pump/LConn1 -- SMAStage3V2HHEXSideFluidTempSensor/LConn1
  SMAHotFluidBufferTempSensor/RConn1 -- SMAHotFluidBufferTempPS/LConn1
  SE_ColdChamberJunction/LConn1 -- ColdFluidBuffer/LConn1 -- ColdFluidBufferTempSensor/LConn1 -- V1ColdInletColdSideFluidTempSensor/LConn1
  V5_cold_return/LConn1 -- SE_ColdChamberJunction/RConn1
  SE_HotChamberJunction/LConn1 -- HotFluidBuffer/LConn1 -- HotFluidBufferTempSensor/LConn1 -- V4HotInletHotSideFluidTempSensor/LConn1 -- 热流体设置/RConn1 -- Solver Configuration/RConn1
  V2_hot_return/LConn1 -- SE_HotChamberJunction/RConn1
  SE_Stage2_PistonPressureSource/LConn1 -- V1_cold_inlet/LConn1
  SE_Stage2_PistonPressureSource/RConn1 -- SE_ColdChamberJunction/RConn2
  SE_Stage4_PistonPressureSource/LConn1 -- V4_hot_inlet/LConn1
  SE_Stage4_PistonPressureSource/RConn1 -- SE_HotChamberJunction/RConn2
  FlowSensor_SMA_stage1_route/RConn2 -- FlowSensor_SMA_stage1_route_PS/LConn1
  FlowSensor_SMA_stage3_route/RConn2 -- FlowSensor_SMA_stage3_route_PS/LConn1
  SMA_V1_SHEX_to_pump/RConn1 -- SMAStage1V1PumpSideFluidTempSensor/LConn1 -- SMA_PumpInletConnectingPipeVolume/LConn1 -- SMA_V2_HHEX_to_pump/RConn1 -- SMAStage3V2PumpSideFluidTempSensor/LConn1
  SMA_PumpInletConnectingPipeVolume/RConn1 -- SMA Pressure Source (TL)/LConn1
  SMA_PumpOutletConnectingPipeVolume/LConn1 -- FlowSensor_SMA_stage13_loop/RConn1 -- SMAStage13PumpOutletFluidTempSensor/LConn1
  FlowSensor_SMA_stage1_route/LConn1 -- SMA_PumpOutletConnectingPipeVolume/RConn1 -- FlowSensor_SMA_stage3_route/LConn1
  FlowSensor_SMA_stage1_route/RConn1 -- SMA_V3_pump_to_heat_path/LConn1
  FlowSensor_SMA_stage3_route/RConn1 -- SMA_V4_pump_to_cool_path/LConn1
  SHEXBufferFluidTempSensor/RConn1 -- SHEXBufferFluidTempPS/LConn1
  SMAStage1V1SHEXSideFluidTempSensor/RConn1 -- SMAStage1V1SHEXSideFluidTempPS/LConn1
  SMAStage1V1PumpSideFluidTempSensor/RConn1 -- SMAStage1V1PumpSideFluidTempPS/LConn1
  SMAStage13PumpOutletFluidTempSensor/RConn1 -- SMAStage13PumpOutletFluidTempPS/LConn1
  SMA/LConn1 -- SMA_V3_pump_to_heat_path/RConn1 -- SMAStage1InletFluidTempSensor/LConn1
  SMAStage1InletFluidTempSensor/RConn1 -- SMAStage1InletFluidTempPS/LConn1
  SMA_V5_SMA_to_SHEX/LConn1 -- SMA/LConn2 -- SMAStage1OutletFluidTempSensor/LConn1
  SMAStage1OutletFluidTempSensor/RConn1 -- SMAStage1OutletFluidTempPS/LConn1
  SHEX/RConn1 -- SMA_V5_SMA_to_SHEX/RConn1 -- SMAStage1V5SHEXSideFluidTempSensor/LConn1
  SMAStage1V5SHEXSideFluidTempSensor/RConn1 -- SMAStage1V5SHEXSideFluidTempPS/LConn1
  SMAStage3V2HHEXSideFluidTempSensor/RConn1 -- SMAStage3V2HHEXSideFluidTempPS/LConn1
  SMAStage3V2PumpSideFluidTempSensor/RConn1 -- SMAStage3V2PumpSideFluidTempPS/LConn1
  SMA/LConn3 -- SMA_V4_pump_to_cool_path/RConn1 -- SMAStage3InletFluidTempSensor/LConn1
  SMAStage3InletFluidTempSensor/RConn1 -- SMAStage3InletFluidTempPS/LConn1
  SMA_V6_SMA_to_HHEX/LConn1 -- SMA/LConn4 -- SMAStage3OutletFluidTempSensor/LConn1
  SMAStage3OutletFluidTempSensor/RConn1 -- SMAStage3OutletFluidTempPS/LConn1
  热端换热器/RConn2 -- SMA_V6_SMA_to_HHEX/RConn1 -- SMAStage3V6HHEXSideFluidTempSensor/LConn1
  SMAStage3V6HHEXSideFluidTempSensor/RConn1 -- SMAStage3V6HHEXSideFluidTempPS/LConn1
